simulink model "heatdrive_ecc_coupled_se21"  (R2025b)
settings: Solver=ode23t  StartTime=0.0  StopTime=10  FixedStep=0.1  MaxStep=0.4  RelTol=1e-2  AbsTol=1e-3
values from neighbouring files (symbols this model uses):
  cold_load_heat_W = 0.0    (= 0)    [Build_Simulink_Exchange_Params.m]
  cold_load_T_init = get_stage_field(stage_config, 'cold_load_T_in', get_stage_field(stage_config,          'chip_T_in', get_option_field(exchange_options, 'cold_load_T_init', get_option_field(exchange_options, 'chip_T_init', 293.0))))    [Build_Simulink_Exchange_Params.m]    (also in Create_Simulink_Exchange_Runtime.m = get_option_field(options, 'cold_load_T_init',          get_o)
  cold_sink_T_init = get_stage_field(stage_config, 'cold_sink_T_in', get_option_field(exchange_options, 'cold_sink_T_init', 293.0))    [Build_Simulink_Exchange_Params.m]    (also in Create_Simulink_Exchange_Runtime.m = get_option_field(options, 'cold_sink_T_init', ambient_T_init)
  hot_sink_T_init = get_stage_field(stage_config, 'hot_sink_T_in', get_option_field(exchange_options, 'hot_sink_T_init', 293.0))    [Build_Simulink_Exchange_Params.m]    (also in Create_Simulink_Exchange_Runtime.m = get_option_field(options, 'hot_sink_T_init', ambient_T_init))
  mdot_cooldown_source_kgps = mdot_target_kgps    [Build_Simulink_Exchange_Params.m]
  mdot_hold_source_kgps = mdot_target_kgps    [Build_Simulink_Exchange_Params.m]
  pressure_pi_bias_MPa = pressure_pi_dp_guess_MPa    [Build_Simulink_Exchange_Params.m]
  pressure_pi_error_filter_tau_s = max(get_option_field(exchange_options, 'pressure_pi_error_filter_tau_s', 0.002), 1.0e-5)    [Build_Simulink_Exchange_Params.m]
  pressure_pi_error_normalization_gain_kgps_inv = 1.0    (= 1)    [Build_Simulink_Exchange_Params.m]
  pressure_pi_max_MPa = pressure_pi_dp_guess_MPa + pressure_pi_margin_MPa    [Build_Simulink_Exchange_Params.m]
  shex_sink_T_init = get_option_field(exchange_options, 'shex_sink_T_init', hot_sink_T_init)    [Build_Simulink_Exchange_Params.m]
undefined symbols (not defined in the file or in its folder): constitutive_sample_time_s, constitutive_state21_initial, se_constitutive_T21_initial, se_pressure_integrator_max_MPa, se_pressure_pi_ki_MPa_per_kgps_s, se_pressure_pi_kp_MPa_per_kgps, se_pressure_pi_min_MPa, se_solver_T_init_21_internal, se_stage2_pressure_integrator_min_MPa, se_stage4_pressure_integrator_min_MPa, sma_constitutive_T21_initial, sma_mdot_stage1_source_kgps, sma_mdot_stage3_source_kgps, sma_pressure_integrator_max_MPa, sma_pressure_integrator_min_MPa, sma_pressure_pi_ki_MPa_per_kgps_s, sma_pressure_pi_kp_MPa_per_kgps, sma_pressure_pi_min_MPa, sma_solver_T_init_21_internal
libraries: fl_lib x484, nesl_utility x232, SimscapeFluids_lib x20
(part 4 of 8)

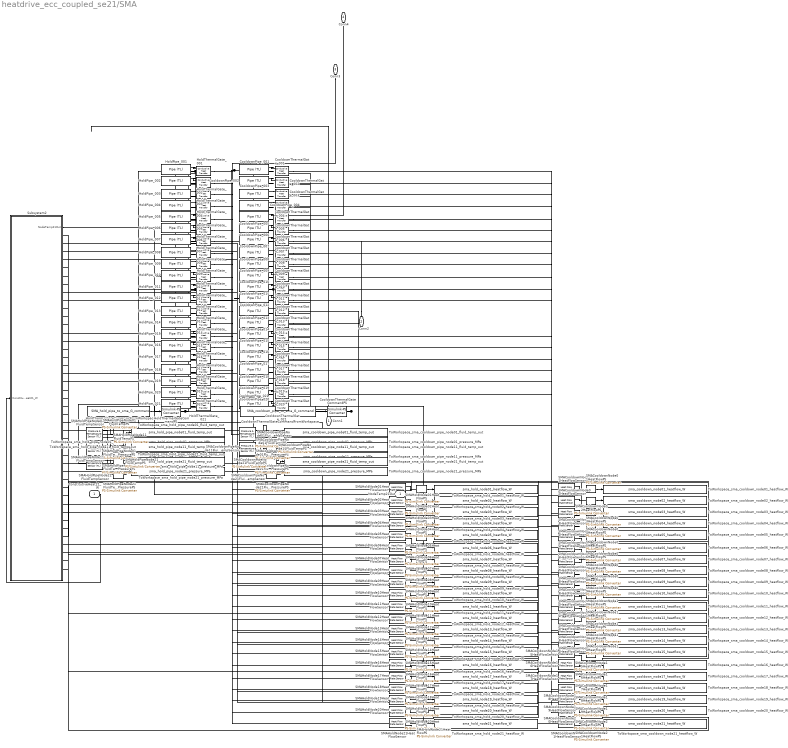
== system heatdrive_ecc_coupled_se21/SMA ==
  ConstitutiveHeat21_W : Inport
  CooldownPipe_001 : fl_lib/Thermal Liquid/Elements/Pipe (TL)  length=sma_article_pipe_segment_l m  area=sma_article_pipe_fa m^2  Dh=sma_article_pipe_Dh m  length_add=0 m  roughness=15e-6 m  Re_lam=2000  Re_tur=4000  shape_factor=64  Nu_lam=sma_article_Nu  dynamic_compressibility=false  inertia=false  p0=1 MPa  T0=sma_cooldown_fluid_T_init K  mdot0=0 kg/s  p_nominal=1 MPa  T_nominal=293.15 K
  CooldownPipe_002 : fl_lib/Thermal Liquid/Elements/Pipe (TL)  length=sma_article_pipe_segment_l m  area=sma_article_pipe_fa m^2  Dh=sma_article_pipe_Dh m  length_add=0 m  roughness=15e-6 m  Re_lam=2000  Re_tur=4000  shape_factor=64  Nu_lam=sma_article_Nu  dynamic_compressibility=false  inertia=false  p0=1 MPa  T0=sma_cooldown_fluid_T_init K  mdot0=0 kg/s  p_nominal=1 MPa  T_nominal=293.15 K
  CooldownPipe_003 : fl_lib/Thermal Liquid/Elements/Pipe (TL)  length=sma_article_pipe_segment_l m  area=sma_article_pipe_fa m^2  Dh=sma_article_pipe_Dh m  length_add=0 m  roughness=15e-6 m  Re_lam=2000  Re_tur=4000  shape_factor=64  Nu_lam=sma_article_Nu  dynamic_compressibility=false  inertia=false  p0=1 MPa  T0=sma_cooldown_fluid_T_init K  mdot0=0 kg/s  p_nominal=1 MPa  T_nominal=293.15 K
  CooldownPipe_004 : fl_lib/Thermal Liquid/Elements/Pipe (TL)  length=sma_article_pipe_segment_l m  area=sma_article_pipe_fa m^2  Dh=sma_article_pipe_Dh m  length_add=0 m  roughness=15e-6 m  Re_lam=2000  Re_tur=4000  shape_factor=64  Nu_lam=sma_article_Nu  dynamic_compressibility=false  inertia=false  p0=1 MPa  T0=sma_cooldown_fluid_T_init K  mdot0=0 kg/s  p_nominal=1 MPa  T_nominal=293.15 K
  CooldownPipe_005 : fl_lib/Thermal Liquid/Elements/Pipe (TL)  length=sma_article_pipe_segment_l m  area=sma_article_pipe_fa m^2  Dh=sma_article_pipe_Dh m  length_add=0 m  roughness=15e-6 m  Re_lam=2000  Re_tur=4000  shape_factor=64  Nu_lam=sma_article_Nu  dynamic_compressibility=false  inertia=false  p0=1 MPa  T0=sma_cooldown_fluid_T_init K  mdot0=0 kg/s  p_nominal=1 MPa  T_nominal=293.15 K
  CooldownPipe_006 : fl_lib/Thermal Liquid/Elements/Pipe (TL)  length=sma_article_pipe_segment_l m  area=sma_article_pipe_fa m^2  Dh=sma_article_pipe_Dh m  length_add=0 m  roughness=15e-6 m  Re_lam=2000  Re_tur=4000  shape_factor=64  Nu_lam=sma_article_Nu  dynamic_compressibility=false  inertia=false  p0=1 MPa  T0=sma_cooldown_fluid_T_init K  mdot0=0 kg/s  p_nominal=1 MPa  T_nominal=293.15 K
  CooldownPipe_007 : fl_lib/Thermal Liquid/Elements/Pipe (TL)  length=sma_article_pipe_segment_l m  area=sma_article_pipe_fa m^2  Dh=sma_article_pipe_Dh m  length_add=0 m  roughness=15e-6 m  Re_lam=2000  Re_tur=4000  shape_factor=64  Nu_lam=sma_article_Nu  dynamic_compressibility=false  inertia=false  p0=1 MPa  T0=sma_cooldown_fluid_T_init K  mdot0=0 kg/s  p_nominal=1 MPa  T_nominal=293.15 K
  CooldownPipe_008 : fl_lib/Thermal Liquid/Elements/Pipe (TL)  length=sma_article_pipe_segment_l m  area=sma_article_pipe_fa m^2  Dh=sma_article_pipe_Dh m  length_add=0 m  roughness=15e-6 m  Re_lam=2000  Re_tur=4000  shape_factor=64  Nu_lam=sma_article_Nu  dynamic_compressibility=false  inertia=false  p0=1 MPa  T0=sma_cooldown_fluid_T_init K  mdot0=0 kg/s  p_nominal=1 MPa  T_nominal=293.15 K
  CooldownPipe_009 : fl_lib/Thermal Liquid/Elements/Pipe (TL)  length=sma_article_pipe_segment_l m  area=sma_article_pipe_fa m^2  Dh=sma_article_pipe_Dh m  length_add=0 m  roughness=15e-6 m  Re_lam=2000  Re_tur=4000  shape_factor=64  Nu_lam=sma_article_Nu  dynamic_compressibility=false  inertia=false  p0=1 MPa  T0=sma_cooldown_fluid_T_init K  mdot0=0 kg/s  p_nominal=1 MPa  T_nominal=293.15 K
  CooldownPipe_010 : fl_lib/Thermal Liquid/Elements/Pipe (TL)  length=sma_article_pipe_segment_l m  area=sma_article_pipe_fa m^2  Dh=sma_article_pipe_Dh m  length_add=0 m  roughness=15e-6 m  Re_lam=2000  Re_tur=4000  shape_factor=64  Nu_lam=sma_article_Nu  dynamic_compressibility=false  inertia=false  p0=1 MPa  T0=sma_cooldown_fluid_T_init K  mdot0=0 kg/s  p_nominal=1 MPa  T_nominal=293.15 K
  CooldownPipe_011 : fl_lib/Thermal Liquid/Elements/Pipe (TL)  length=sma_article_pipe_segment_l m  area=sma_article_pipe_fa m^2  Dh=sma_article_pipe_Dh m  length_add=0 m  roughness=15e-6 m  Re_lam=2000  Re_tur=4000  shape_factor=64  Nu_lam=sma_article_Nu  dynamic_compressibility=false  inertia=false  p0=1 MPa  T0=sma_cooldown_fluid_T_init K  mdot0=0 kg/s  p_nominal=1 MPa  T_nominal=293.15 K
  CooldownPipe_012 : fl_lib/Thermal Liquid/Elements/Pipe (TL)  length=sma_article_pipe_segment_l m  area=sma_article_pipe_fa m^2  Dh=sma_article_pipe_Dh m  length_add=0 m  roughness=15e-6 m  Re_lam=2000  Re_tur=4000  shape_factor=64  Nu_lam=sma_article_Nu  dynamic_compressibility=false  inertia=false  p0=1 MPa  T0=sma_cooldown_fluid_T_init K  mdot0=0 kg/s  p_nominal=1 MPa  T_nominal=293.15 K
  CooldownPipe_013 : fl_lib/Thermal Liquid/Elements/Pipe (TL)  length=sma_article_pipe_segment_l m  area=sma_article_pipe_fa m^2  Dh=sma_article_pipe_Dh m  length_add=0 m  roughness=15e-6 m  Re_lam=2000  Re_tur=4000  shape_factor=64  Nu_lam=sma_article_Nu  dynamic_compressibility=false  inertia=false  p0=1 MPa  T0=sma_cooldown_fluid_T_init K  mdot0=0 kg/s  p_nominal=1 MPa  T_nominal=293.15 K
  CooldownPipe_014 : fl_lib/Thermal Liquid/Elements/Pipe (TL)  length=sma_article_pipe_segment_l m  area=sma_article_pipe_fa m^2  Dh=sma_article_pipe_Dh m  length_add=0 m  roughness=15e-6 m  Re_lam=2000  Re_tur=4000  shape_factor=64  Nu_lam=sma_article_Nu  dynamic_compressibility=false  inertia=false  p0=1 MPa  T0=sma_cooldown_fluid_T_init K  mdot0=0 kg/s  p_nominal=1 MPa  T_nominal=293.15 K
  CooldownPipe_015 : fl_lib/Thermal Liquid/Elements/Pipe (TL)  length=sma_article_pipe_segment_l m  area=sma_article_pipe_fa m^2  Dh=sma_article_pipe_Dh m  length_add=0 m  roughness=15e-6 m  Re_lam=2000  Re_tur=4000  shape_factor=64  Nu_lam=sma_article_Nu  dynamic_compressibility=false  inertia=false  p0=1 MPa  T0=sma_cooldown_fluid_T_init K  mdot0=0 kg/s  p_nominal=1 MPa  T_nominal=293.15 K
  CooldownPipe_016 : fl_lib/Thermal Liquid/Elements/Pipe (TL)  length=sma_article_pipe_segment_l m  area=sma_article_pipe_fa m^2  Dh=sma_article_pipe_Dh m  length_add=0 m  roughness=15e-6 m  Re_lam=2000  Re_tur=4000  shape_factor=64  Nu_lam=sma_article_Nu  dynamic_compressibility=false  inertia=false  p0=1 MPa  T0=sma_cooldown_fluid_T_init K  mdot0=0 kg/s  p_nominal=1 MPa  T_nominal=293.15 K
  CooldownPipe_017 : fl_lib/Thermal Liquid/Elements/Pipe (TL)  length=sma_article_pipe_segment_l m  area=sma_article_pipe_fa m^2  Dh=sma_article_pipe_Dh m  length_add=0 m  roughness=15e-6 m  Re_lam=2000  Re_tur=4000  shape_factor=64  Nu_lam=sma_article_Nu  dynamic_compressibility=false  inertia=false  p0=1 MPa  T0=sma_cooldown_fluid_T_init K  mdot0=0 kg/s  p_nominal=1 MPa  T_nominal=293.15 K
  CooldownPipe_018 : fl_lib/Thermal Liquid/Elements/Pipe (TL)  length=sma_article_pipe_segment_l m  area=sma_article_pipe_fa m^2  Dh=sma_article_pipe_Dh m  length_add=0 m  roughness=15e-6 m  Re_lam=2000  Re_tur=4000  shape_factor=64  Nu_lam=sma_article_Nu  dynamic_compressibility=false  inertia=false  p0=1 MPa  T0=sma_cooldown_fluid_T_init K  mdot0=0 kg/s  p_nominal=1 MPa  T_nominal=293.15 K
  CooldownPipe_019 : fl_lib/Thermal Liquid/Elements/Pipe (TL)  length=sma_article_pipe_segment_l m  area=sma_article_pipe_fa m^2  Dh=sma_article_pipe_Dh m  length_add=0 m  roughness=15e-6 m  Re_lam=2000  Re_tur=4000  shape_factor=64  Nu_lam=sma_article_Nu  dynamic_compressibility=false  inertia=false  p0=1 MPa  T0=sma_cooldown_fluid_T_init K  mdot0=0 kg/s  p_nominal=1 MPa  T_nominal=293.15 K
  CooldownPipe_020 : fl_lib/Thermal Liquid/Elements/Pipe (TL)  length=sma_article_pipe_segment_l m  area=sma_article_pipe_fa m^2  Dh=sma_article_pipe_Dh m  length_add=0 m  roughness=15e-6 m  Re_lam=2000  Re_tur=4000  shape_factor=64  Nu_lam=sma_article_Nu  dynamic_compressibility=false  inertia=false  p0=1 MPa  T0=sma_cooldown_fluid_T_init K  mdot0=0 kg/s  p_nominal=1 MPa  T_nominal=293.15 K
  CooldownPipe_021 : fl_lib/Thermal Liquid/Elements/Pipe (TL)  length=sma_article_pipe_segment_l m  area=sma_article_pipe_fa m^2  Dh=sma_article_pipe_Dh m  length_add=0 m  roughness=15e-6 m  Re_lam=2000  Re_tur=4000  shape_factor=64  Nu_lam=sma_article_Nu  dynamic_compressibility=false  inertia=false  p0=1 MPa  T0=sma_cooldown_fluid_T_init K  mdot0=0 kg/s  p_nominal=1 MPa  T_nominal=293.15 K
  CooldownThermalGateCommandFromWorkspace : FromWorkspace  VariableName=SMA_cooldown_pipe_to_sma_G_command  Interpolate=off  OutputAfterFinalValue=Holding final value
  CooldownThermalGateCommandPS : nesl_utility/Simulink-PS Converter  PhysicalDomain=network_engine_domain  SubClassName=ps_input  LeftPortType=input  RightPortType=output  PseudoPeriodic=off  Frequencies=[]  NoiseDistribution=none  NoiseParameters=[]  Unit=W/(K*m)  AffineConversion=off  FilteringAndDerivatives=provide  SimscapeFilterOrder=1  InputFilterTimeConstant=0.001  UdotUserProvided=0
  CooldownThermalGate_001 : fl_lib/Thermal/Thermal Elements/Conductive Heat Transfer  thermal_type=foundation.enum.ConstantVariableTabulated.Variable  wall_geometry=foundation.enum.ConductionWallGeometry.Planar  area=sma_pipe_fa m^2  thickness=1 m  d_in=0.05 m  d_out=0.1 m  L=1 m  th_cond_min=thermal_gate_min_conductivity_W_per_mK W/(K*m)  th_cond=sma_cooldown_pipe_to_sma_G_W_per_K W/(K*m)  th_cond_TLU=[413, 401, 392, 383, 371, 357, 342] W/(K*m)  temp_TLU=[200, 273, 400, 600, 800, 1000, 1200] K  T_specify=off  T_priority=None  T=0 K  T_nominal_specify=off  T_nominal_value=1  T_nominal_unit=K  Q_specify=off  Q_priority=None  Q=0 W  Q_nominal_specify=off  Q_nominal_value=1  Q_nominal_unit=W
      settings: InternalSimscapePortConfiguration="{\"Bottom\":[],\"Left\":[{\"id\":\"A\",\"label\":\"A\",\"type\":\"foundation.thermal.thermal\"},{\"id\":\"var_th_cond\",\"label\":\"K\",\"type\":\"input\"}],\"Right\":[{\"id\":\"B\",\"label\":\"B\",\"type\":\"foundation.thermal.thermal\"}],\"Top\":[]}"
  CooldownThermalGate_002 : fl_lib/Thermal/Thermal Elements/Conductive Heat Transfer  thermal_type=foundation.enum.ConstantVariableTabulated.Variable  wall_geometry=foundation.enum.ConductionWallGeometry.Planar  area=sma_pipe_fa m^2  thickness=1 m  d_in=0.05 m  d_out=0.1 m  L=1 m  th_cond_min=thermal_gate_min_conductivity_W_per_mK W/(K*m)  th_cond=sma_cooldown_pipe_to_sma_G_W_per_K W/(K*m)  th_cond_TLU=[413, 401, 392, 383, 371, 357, 342] W/(K*m)  temp_TLU=[200, 273, 400, 600, 800, 1000, 1200] K  T_specify=off  T_priority=None  T=0 K  T_nominal_specify=off  T_nominal_value=1  T_nominal_unit=K  Q_specify=off  Q_priority=None  Q=0 W  Q_nominal_specify=off  Q_nominal_value=1  Q_nominal_unit=W
      settings: InternalSimscapePortConfiguration="{\"Bottom\":[],\"Left\":[{\"id\":\"A\",\"label\":\"A\",\"type\":\"foundation.thermal.thermal\"},{\"id\":\"var_th_cond\",\"label\":\"K\",\"type\":\"input\"}],\"Right\":[{\"id\":\"B\",\"label\":\"B\",\"type\":\"foundation.thermal.thermal\"}],\"Top\":[]}"
  CooldownThermalGate_003 : fl_lib/Thermal/Thermal Elements/Conductive Heat Transfer  thermal_type=foundation.enum.ConstantVariableTabulated.Variable  wall_geometry=foundation.enum.ConductionWallGeometry.Planar  area=sma_pipe_fa m^2  thickness=1 m  d_in=0.05 m  d_out=0.1 m  L=1 m  th_cond_min=thermal_gate_min_conductivity_W_per_mK W/(K*m)  th_cond=sma_cooldown_pipe_to_sma_G_W_per_K W/(K*m)  th_cond_TLU=[413, 401, 392, 383, 371, 357, 342] W/(K*m)  temp_TLU=[200, 273, 400, 600, 800, 1000, 1200] K  T_specify=off  T_priority=None  T=0 K  T_nominal_specify=off  T_nominal_value=1  T_nominal_unit=K  Q_specify=off  Q_priority=None  Q=0 W  Q_nominal_specify=off  Q_nominal_value=1  Q_nominal_unit=W
      settings: InternalSimscapePortConfiguration="{\"Bottom\":[],\"Left\":[{\"id\":\"A\",\"label\":\"A\",\"type\":\"foundation.thermal.thermal\"},{\"id\":\"var_th_cond\",\"label\":\"K\",\"type\":\"input\"}],\"Right\":[{\"id\":\"B\",\"label\":\"B\",\"type\":\"foundation.thermal.thermal\"}],\"Top\":[]}"
  CooldownThermalGate_004 : fl_lib/Thermal/Thermal Elements/Conductive Heat Transfer  thermal_type=foundation.enum.ConstantVariableTabulated.Variable  wall_geometry=foundation.enum.ConductionWallGeometry.Planar  area=sma_pipe_fa m^2  thickness=1 m  d_in=0.05 m  d_out=0.1 m  L=1 m  th_cond_min=thermal_gate_min_conductivity_W_per_mK W/(K*m)  th_cond=sma_cooldown_pipe_to_sma_G_W_per_K W/(K*m)  th_cond_TLU=[413, 401, 392, 383, 371, 357, 342] W/(K*m)  temp_TLU=[200, 273, 400, 600, 800, 1000, 1200] K  T_specify=off  T_priority=None  T=0 K  T_nominal_specify=off  T_nominal_value=1  T_nominal_unit=K  Q_specify=off  Q_priority=None  Q=0 W  Q_nominal_specify=off  Q_nominal_value=1  Q_nominal_unit=W
      settings: InternalSimscapePortConfiguration="{\"Bottom\":[],\"Left\":[{\"id\":\"A\",\"label\":\"A\",\"type\":\"foundation.thermal.thermal\"},{\"id\":\"var_th_cond\",\"label\":\"K\",\"type\":\"input\"}],\"Right\":[{\"id\":\"B\",\"label\":\"B\",\"type\":\"foundation.thermal.thermal\"}],\"Top\":[]}"
  CooldownThermalGate_005 : fl_lib/Thermal/Thermal Elements/Conductive Heat Transfer  thermal_type=foundation.enum.ConstantVariableTabulated.Variable  wall_geometry=foundation.enum.ConductionWallGeometry.Planar  area=sma_pipe_fa m^2  thickness=1 m  d_in=0.05 m  d_out=0.1 m  L=1 m  th_cond_min=thermal_gate_min_conductivity_W_per_mK W/(K*m)  th_cond=sma_cooldown_pipe_to_sma_G_W_per_K W/(K*m)  th_cond_TLU=[413, 401, 392, 383, 371, 357, 342] W/(K*m)  temp_TLU=[200, 273, 400, 600, 800, 1000, 1200] K  T_specify=off  T_priority=None  T=0 K  T_nominal_specify=off  T_nominal_value=1  T_nominal_unit=K  Q_specify=off  Q_priority=None  Q=0 W  Q_nominal_specify=off  Q_nominal_value=1  Q_nominal_unit=W
      settings: InternalSimscapePortConfiguration="{\"Bottom\":[],\"Left\":[{\"id\":\"A\",\"label\":\"A\",\"type\":\"foundation.thermal.thermal\"},{\"id\":\"var_th_cond\",\"label\":\"K\",\"type\":\"input\"}],\"Right\":[{\"id\":\"B\",\"label\":\"B\",\"type\":\"foundation.thermal.thermal\"}],\"Top\":[]}"
  CooldownThermalGate_006 : fl_lib/Thermal/Thermal Elements/Conductive Heat Transfer  thermal_type=foundation.enum.ConstantVariableTabulated.Variable  wall_geometry=foundation.enum.ConductionWallGeometry.Planar  area=sma_pipe_fa m^2  thickness=1 m  d_in=0.05 m  d_out=0.1 m  L=1 m  th_cond_min=thermal_gate_min_conductivity_W_per_mK W/(K*m)  th_cond=sma_cooldown_pipe_to_sma_G_W_per_K W/(K*m)  th_cond_TLU=[413, 401, 392, 383, 371, 357, 342] W/(K*m)  temp_TLU=[200, 273, 400, 600, 800, 1000, 1200] K  T_specify=off  T_priority=None  T=0 K  T_nominal_specify=off  T_nominal_value=1  T_nominal_unit=K  Q_specify=off  Q_priority=None  Q=0 W  Q_nominal_specify=off  Q_nominal_value=1  Q_nominal_unit=W
      settings: InternalSimscapePortConfiguration="{\"Bottom\":[],\"Left\":[{\"id\":\"A\",\"label\":\"A\",\"type\":\"foundation.thermal.thermal\"},{\"id\":\"var_th_cond\",\"label\":\"K\",\"type\":\"input\"}],\"Right\":[{\"id\":\"B\",\"label\":\"B\",\"type\":\"foundation.thermal.thermal\"}],\"Top\":[]}"
  CooldownThermalGate_007 : fl_lib/Thermal/Thermal Elements/Conductive Heat Transfer  thermal_type=foundation.enum.ConstantVariableTabulated.Variable  wall_geometry=foundation.enum.ConductionWallGeometry.Planar  area=sma_pipe_fa m^2  thickness=1 m  d_in=0.05 m  d_out=0.1 m  L=1 m  th_cond_min=thermal_gate_min_conductivity_W_per_mK W/(K*m)  th_cond=sma_cooldown_pipe_to_sma_G_W_per_K W/(K*m)  th_cond_TLU=[413, 401, 392, 383, 371, 357, 342] W/(K*m)  temp_TLU=[200, 273, 400, 600, 800, 1000, 1200] K  T_specify=off  T_priority=None  T=0 K  T_nominal_specify=off  T_nominal_value=1  T_nominal_unit=K  Q_specify=off  Q_priority=None  Q=0 W  Q_nominal_specify=off  Q_nominal_value=1  Q_nominal_unit=W
      settings: InternalSimscapePortConfiguration="{\"Bottom\":[],\"Left\":[{\"id\":\"A\",\"label\":\"A\",\"type\":\"foundation.thermal.thermal\"},{\"id\":\"var_th_cond\",\"label\":\"K\",\"type\":\"input\"}],\"Right\":[{\"id\":\"B\",\"label\":\"B\",\"type\":\"foundation.thermal.thermal\"}],\"Top\":[]}"
  CooldownThermalGate_008 : fl_lib/Thermal/Thermal Elements/Conductive Heat Transfer  thermal_type=foundation.enum.ConstantVariableTabulated.Variable  wall_geometry=foundation.enum.ConductionWallGeometry.Planar  area=sma_pipe_fa m^2  thickness=1 m  d_in=0.05 m  d_out=0.1 m  L=1 m  th_cond_min=thermal_gate_min_conductivity_W_per_mK W/(K*m)  th_cond=sma_cooldown_pipe_to_sma_G_W_per_K W/(K*m)  th_cond_TLU=[413, 401, 392, 383, 371, 357, 342] W/(K*m)  temp_TLU=[200, 273, 400, 600, 800, 1000, 1200] K  T_specify=off  T_priority=None  T=0 K  T_nominal_specify=off  T_nominal_value=1  T_nominal_unit=K  Q_specify=off  Q_priority=None  Q=0 W  Q_nominal_specify=off  Q_nominal_value=1  Q_nominal_unit=W
      settings: InternalSimscapePortConfiguration="{\"Bottom\":[],\"Left\":[{\"id\":\"A\",\"label\":\"A\",\"type\":\"foundation.thermal.thermal\"},{\"id\":\"var_th_cond\",\"label\":\"K\",\"type\":\"input\"}],\"Right\":[{\"id\":\"B\",\"label\":\"B\",\"type\":\"foundation.thermal.thermal\"}],\"Top\":[]}"
  CooldownThermalGate_009 : fl_lib/Thermal/Thermal Elements/Conductive Heat Transfer  thermal_type=foundation.enum.ConstantVariableTabulated.Variable  wall_geometry=foundation.enum.ConductionWallGeometry.Planar  area=sma_pipe_fa m^2  thickness=1 m  d_in=0.05 m  d_out=0.1 m  L=1 m  th_cond_min=thermal_gate_min_conductivity_W_per_mK W/(K*m)  th_cond=sma_cooldown_pipe_to_sma_G_W_per_K W/(K*m)  th_cond_TLU=[413, 401, 392, 383, 371, 357, 342] W/(K*m)  temp_TLU=[200, 273, 400, 600, 800, 1000, 1200] K  T_specify=off  T_priority=None  T=0 K  T_nominal_specify=off  T_nominal_value=1  T_nominal_unit=K  Q_specify=off  Q_priority=None  Q=0 W  Q_nominal_specify=off  Q_nominal_value=1  Q_nominal_unit=W
      settings: InternalSimscapePortConfiguration="{\"Bottom\":[],\"Left\":[{\"id\":\"A\",\"label\":\"A\",\"type\":\"foundation.thermal.thermal\"},{\"id\":\"var_th_cond\",\"label\":\"K\",\"type\":\"input\"}],\"Right\":[{\"id\":\"B\",\"label\":\"B\",\"type\":\"foundation.thermal.thermal\"}],\"Top\":[]}"
  CooldownThermalGate_010 : fl_lib/Thermal/Thermal Elements/Conductive Heat Transfer  thermal_type=foundation.enum.ConstantVariableTabulated.Variable  wall_geometry=foundation.enum.ConductionWallGeometry.Planar  area=sma_pipe_fa m^2  thickness=1 m  d_in=0.05 m  d_out=0.1 m  L=1 m  th_cond_min=thermal_gate_min_conductivity_W_per_mK W/(K*m)  th_cond=sma_cooldown_pipe_to_sma_G_W_per_K W/(K*m)  th_cond_TLU=[413, 401, 392, 383, 371, 357, 342] W/(K*m)  temp_TLU=[200, 273, 400, 600, 800, 1000, 1200] K  T_specify=off  T_priority=None  T=0 K  T_nominal_specify=off  T_nominal_value=1  T_nominal_unit=K  Q_specify=off  Q_priority=None  Q=0 W  Q_nominal_specify=off  Q_nominal_value=1  Q_nominal_unit=W
      settings: InternalSimscapePortConfiguration="{\"Bottom\":[],\"Left\":[{\"id\":\"A\",\"label\":\"A\",\"type\":\"foundation.thermal.thermal\"},{\"id\":\"var_th_cond\",\"label\":\"K\",\"type\":\"input\"}],\"Right\":[{\"id\":\"B\",\"label\":\"B\",\"type\":\"foundation.thermal.thermal\"}],\"Top\":[]}"
  CooldownThermalGate_011 : fl_lib/Thermal/Thermal Elements/Conductive Heat Transfer  thermal_type=foundation.enum.ConstantVariableTabulated.Variable  wall_geometry=foundation.enum.ConductionWallGeometry.Planar  area=sma_pipe_fa m^2  thickness=1 m  d_in=0.05 m  d_out=0.1 m  L=1 m  th_cond_min=thermal_gate_min_conductivity_W_per_mK W/(K*m)  th_cond=sma_cooldown_pipe_to_sma_G_W_per_K W/(K*m)  th_cond_TLU=[413, 401, 392, 383, 371, 357, 342] W/(K*m)  temp_TLU=[200, 273, 400, 600, 800, 1000, 1200] K  T_specify=off  T_priority=None  T=0 K  T_nominal_specify=off  T_nominal_value=1  T_nominal_unit=K  Q_specify=off  Q_priority=None  Q=0 W  Q_nominal_specify=off  Q_nominal_value=1  Q_nominal_unit=W
      settings: InternalSimscapePortConfiguration="{\"Bottom\":[],\"Left\":[{\"id\":\"A\",\"label\":\"A\",\"type\":\"foundation.thermal.thermal\"},{\"id\":\"var_th_cond\",\"label\":\"K\",\"type\":\"input\"}],\"Right\":[{\"id\":\"B\",\"label\":\"B\",\"type\":\"foundation.thermal.thermal\"}],\"Top\":[]}"
  CooldownThermalGate_012 : fl_lib/Thermal/Thermal Elements/Conductive Heat Transfer  thermal_type=foundation.enum.ConstantVariableTabulated.Variable  wall_geometry=foundation.enum.ConductionWallGeometry.Planar  area=sma_pipe_fa m^2  thickness=1 m  d_in=0.05 m  d_out=0.1 m  L=1 m  th_cond_min=thermal_gate_min_conductivity_W_per_mK W/(K*m)  th_cond=sma_cooldown_pipe_to_sma_G_W_per_K W/(K*m)  th_cond_TLU=[413, 401, 392, 383, 371, 357, 342] W/(K*m)  temp_TLU=[200, 273, 400, 600, 800, 1000, 1200] K  T_specify=off  T_priority=None  T=0 K  T_nominal_specify=off  T_nominal_value=1  T_nominal_unit=K  Q_specify=off  Q_priority=None  Q=0 W  Q_nominal_specify=off  Q_nominal_value=1  Q_nominal_unit=W
      settings: InternalSimscapePortConfiguration="{\"Bottom\":[],\"Left\":[{\"id\":\"A\",\"label\":\"A\",\"type\":\"foundation.thermal.thermal\"},{\"id\":\"var_th_cond\",\"label\":\"K\",\"type\":\"input\"}],\"Right\":[{\"id\":\"B\",\"label\":\"B\",\"type\":\"foundation.thermal.thermal\"}],\"Top\":[]}"
  CooldownThermalGate_013 : fl_lib/Thermal/Thermal Elements/Conductive Heat Transfer  thermal_type=foundation.enum.ConstantVariableTabulated.Variable  wall_geometry=foundation.enum.ConductionWallGeometry.Planar  area=sma_pipe_fa m^2  thickness=1 m  d_in=0.05 m  d_out=0.1 m  L=1 m  th_cond_min=thermal_gate_min_conductivity_W_per_mK W/(K*m)  th_cond=sma_cooldown_pipe_to_sma_G_W_per_K W/(K*m)  th_cond_TLU=[413, 401, 392, 383, 371, 357, 342] W/(K*m)  temp_TLU=[200, 273, 400, 600, 800, 1000, 1200] K  T_specify=off  T_priority=None  T=0 K  T_nominal_specify=off  T_nominal_value=1  T_nominal_unit=K  Q_specify=off  Q_priority=None  Q=0 W  Q_nominal_specify=off  Q_nominal_value=1  Q_nominal_unit=W
      settings: InternalSimscapePortConfiguration="{\"Bottom\":[],\"Left\":[{\"id\":\"A\",\"label\":\"A\",\"type\":\"foundation.thermal.thermal\"},{\"id\":\"var_th_cond\",\"label\":\"K\",\"type\":\"input\"}],\"Right\":[{\"id\":\"B\",\"label\":\"B\",\"type\":\"foundation.thermal.thermal\"}],\"Top\":[]}"
  CooldownThermalGate_014 : fl_lib/Thermal/Thermal Elements/Conductive Heat Transfer  thermal_type=foundation.enum.ConstantVariableTabulated.Variable  wall_geometry=foundation.enum.ConductionWallGeometry.Planar  area=sma_pipe_fa m^2  thickness=1 m  d_in=0.05 m  d_out=0.1 m  L=1 m  th_cond_min=thermal_gate_min_conductivity_W_per_mK W/(K*m)  th_cond=sma_cooldown_pipe_to_sma_G_W_per_K W/(K*m)  th_cond_TLU=[413, 401, 392, 383, 371, 357, 342] W/(K*m)  temp_TLU=[200, 273, 400, 600, 800, 1000, 1200] K  T_specify=off  T_priority=None  T=0 K  T_nominal_specify=off  T_nominal_value=1  T_nominal_unit=K  Q_specify=off  Q_priority=None  Q=0 W  Q_nominal_specify=off  Q_nominal_value=1  Q_nominal_unit=W
      settings: InternalSimscapePortConfiguration="{\"Bottom\":[],\"Left\":[{\"id\":\"A\",\"label\":\"A\",\"type\":\"foundation.thermal.thermal\"},{\"id\":\"var_th_cond\",\"label\":\"K\",\"type\":\"input\"}],\"Right\":[{\"id\":\"B\",\"label\":\"B\",\"type\":\"foundation.thermal.thermal\"}],\"Top\":[]}"
  CooldownThermalGate_015 : fl_lib/Thermal/Thermal Elements/Conductive Heat Transfer  thermal_type=foundation.enum.ConstantVariableTabulated.Variable  wall_geometry=foundation.enum.ConductionWallGeometry.Planar  area=sma_pipe_fa m^2  thickness=1 m  d_in=0.05 m  d_out=0.1 m  L=1 m  th_cond_min=thermal_gate_min_conductivity_W_per_mK W/(K*m)  th_cond=sma_cooldown_pipe_to_sma_G_W_per_K W/(K*m)  th_cond_TLU=[413, 401, 392, 383, 371, 357, 342] W/(K*m)  temp_TLU=[200, 273, 400, 600, 800, 1000, 1200] K  T_specify=off  T_priority=None  T=0 K  T_nominal_specify=off  T_nominal_value=1  T_nominal_unit=K  Q_specify=off  Q_priority=None  Q=0 W  Q_nominal_specify=off  Q_nominal_value=1  Q_nominal_unit=W
      settings: InternalSimscapePortConfiguration="{\"Bottom\":[],\"Left\":[{\"id\":\"A\",\"label\":\"A\",\"type\":\"foundation.thermal.thermal\"},{\"id\":\"var_th_cond\",\"label\":\"K\",\"type\":\"input\"}],\"Right\":[{\"id\":\"B\",\"label\":\"B\",\"type\":\"foundation.thermal.thermal\"}],\"Top\":[]}"
  CooldownThermalGate_016 : fl_lib/Thermal/Thermal Elements/Conductive Heat Transfer  thermal_type=foundation.enum.ConstantVariableTabulated.Variable  wall_geometry=foundation.enum.ConductionWallGeometry.Planar  area=sma_pipe_fa m^2  thickness=1 m  d_in=0.05 m  d_out=0.1 m  L=1 m  th_cond_min=thermal_gate_min_conductivity_W_per_mK W/(K*m)  th_cond=sma_cooldown_pipe_to_sma_G_W_per_K W/(K*m)  th_cond_TLU=[413, 401, 392, 383, 371, 357, 342] W/(K*m)  temp_TLU=[200, 273, 400, 600, 800, 1000, 1200] K  T_specify=off  T_priority=None  T=0 K  T_nominal_specify=off  T_nominal_value=1  T_nominal_unit=K  Q_specify=off  Q_priority=None  Q=0 W  Q_nominal_specify=off  Q_nominal_value=1  Q_nominal_unit=W
      settings: InternalSimscapePortConfiguration="{\"Bottom\":[],\"Left\":[{\"id\":\"A\",\"label\":\"A\",\"type\":\"foundation.thermal.thermal\"},{\"id\":\"var_th_cond\",\"label\":\"K\",\"type\":\"input\"}],\"Right\":[{\"id\":\"B\",\"label\":\"B\",\"type\":\"foundation.thermal.thermal\"}],\"Top\":[]}"
  CooldownThermalGate_017 : fl_lib/Thermal/Thermal Elements/Conductive Heat Transfer  thermal_type=foundation.enum.ConstantVariableTabulated.Variable  wall_geometry=foundation.enum.ConductionWallGeometry.Planar  area=sma_pipe_fa m^2  thickness=1 m  d_in=0.05 m  d_out=0.1 m  L=1 m  th_cond_min=thermal_gate_min_conductivity_W_per_mK W/(K*m)  th_cond=sma_cooldown_pipe_to_sma_G_W_per_K W/(K*m)  th_cond_TLU=[413, 401, 392, 383, 371, 357, 342] W/(K*m)  temp_TLU=[200, 273, 400, 600, 800, 1000, 1200] K  T_specify=off  T_priority=None  T=0 K  T_nominal_specify=off  T_nominal_value=1  T_nominal_unit=K  Q_specify=off  Q_priority=None  Q=0 W  Q_nominal_specify=off  Q_nominal_value=1  Q_nominal_unit=W
      settings: InternalSimscapePortConfiguration="{\"Bottom\":[],\"Left\":[{\"id\":\"A\",\"label\":\"A\",\"type\":\"foundation.thermal.thermal\"},{\"id\":\"var_th_cond\",\"label\":\"K\",\"type\":\"input\"}],\"Right\":[{\"id\":\"B\",\"label\":\"B\",\"type\":\"foundation.thermal.thermal\"}],\"Top\":[]}"
  CooldownThermalGate_018 : fl_lib/Thermal/Thermal Elements/Conductive Heat Transfer  thermal_type=foundation.enum.ConstantVariableTabulated.Variable  wall_geometry=foundation.enum.ConductionWallGeometry.Planar  area=sma_pipe_fa m^2  thickness=1 m  d_in=0.05 m  d_out=0.1 m  L=1 m  th_cond_min=thermal_gate_min_conductivity_W_per_mK W/(K*m)  th_cond=sma_cooldown_pipe_to_sma_G_W_per_K W/(K*m)  th_cond_TLU=[413, 401, 392, 383, 371, 357, 342] W/(K*m)  temp_TLU=[200, 273, 400, 600, 800, 1000, 1200] K  T_specify=off  T_priority=None  T=0 K  T_nominal_specify=off  T_nominal_value=1  T_nominal_unit=K  Q_specify=off  Q_priority=None  Q=0 W  Q_nominal_specify=off  Q_nominal_value=1  Q_nominal_unit=W
      settings: InternalSimscapePortConfiguration="{\"Bottom\":[],\"Left\":[{\"id\":\"A\",\"label\":\"A\",\"type\":\"foundation.thermal.thermal\"},{\"id\":\"var_th_cond\",\"label\":\"K\",\"type\":\"input\"}],\"Right\":[{\"id\":\"B\",\"label\":\"B\",\"type\":\"foundation.thermal.thermal\"}],\"Top\":[]}"
  CooldownThermalGate_019 : fl_lib/Thermal/Thermal Elements/Conductive Heat Transfer  thermal_type=foundation.enum.ConstantVariableTabulated.Variable  wall_geometry=foundation.enum.ConductionWallGeometry.Planar  area=sma_pipe_fa m^2  thickness=1 m  d_in=0.05 m  d_out=0.1 m  L=1 m  th_cond_min=thermal_gate_min_conductivity_W_per_mK W/(K*m)  th_cond=sma_cooldown_pipe_to_sma_G_W_per_K W/(K*m)  th_cond_TLU=[413, 401, 392, 383, 371, 357, 342] W/(K*m)  temp_TLU=[200, 273, 400, 600, 800, 1000, 1200] K  T_specify=off  T_priority=None  T=0 K  T_nominal_specify=off  T_nominal_value=1  T_nominal_unit=K  Q_specify=off  Q_priority=None  Q=0 W  Q_nominal_specify=off  Q_nominal_value=1  Q_nominal_unit=W
      settings: InternalSimscapePortConfiguration="{\"Bottom\":[],\"Left\":[{\"id\":\"A\",\"label\":\"A\",\"type\":\"foundation.thermal.thermal\"},{\"id\":\"var_th_cond\",\"label\":\"K\",\"type\":\"input\"}],\"Right\":[{\"id\":\"B\",\"label\":\"B\",\"type\":\"foundation.thermal.thermal\"}],\"Top\":[]}"
  CooldownThermalGate_020 : fl_lib/Thermal/Thermal Elements/Conductive Heat Transfer  thermal_type=foundation.enum.ConstantVariableTabulated.Variable  wall_geometry=foundation.enum.ConductionWallGeometry.Planar  area=sma_pipe_fa m^2  thickness=1 m  d_in=0.05 m  d_out=0.1 m  L=1 m  th_cond_min=thermal_gate_min_conductivity_W_per_mK W/(K*m)  th_cond=sma_cooldown_pipe_to_sma_G_W_per_K W/(K*m)  th_cond_TLU=[413, 401, 392, 383, 371, 357, 342] W/(K*m)  temp_TLU=[200, 273, 400, 600, 800, 1000, 1200] K  T_specify=off  T_priority=None  T=0 K  T_nominal_specify=off  T_nominal_value=1  T_nominal_unit=K  Q_specify=off  Q_priority=None  Q=0 W  Q_nominal_specify=off  Q_nominal_value=1  Q_nominal_unit=W
      settings: InternalSimscapePortConfiguration="{\"Bottom\":[],\"Left\":[{\"id\":\"A\",\"label\":\"A\",\"type\":\"foundation.thermal.thermal\"},{\"id\":\"var_th_cond\",\"label\":\"K\",\"type\":\"input\"}],\"Right\":[{\"id\":\"B\",\"label\":\"B\",\"type\":\"foundation.thermal.thermal\"}],\"Top\":[]}"
  CooldownThermalGate_021 : fl_lib/Thermal/Thermal Elements/Conductive Heat Transfer  thermal_type=foundation.enum.ConstantVariableTabulated.Variable  wall_geometry=foundation.enum.ConductionWallGeometry.Planar  area=sma_pipe_fa m^2  thickness=1 m  d_in=0.05 m  d_out=0.1 m  L=1 m  th_cond_min=thermal_gate_min_conductivity_W_per_mK W/(K*m)  th_cond=sma_cooldown_pipe_to_sma_G_W_per_K W/(K*m)  th_cond_TLU=[413, 401, 392, 383, 371, 357, 342] W/(K*m)  temp_TLU=[200, 273, 400, 600, 800, 1000, 1200] K  T_specify=off  T_priority=None  T=0 K  T_nominal_specify=off  T_nominal_value=1  T_nominal_unit=K  Q_specify=off  Q_priority=None  Q=0 W  Q_nominal_specify=off  Q_nominal_value=1  Q_nominal_unit=W
      settings: InternalSimscapePortConfiguration="{\"Bottom\":[],\"Left\":[{\"id\":\"A\",\"label\":\"A\",\"type\":\"foundation.thermal.thermal\"},{\"id\":\"var_th_cond\",\"label\":\"K\",\"type\":\"input\"}],\"Right\":[{\"id\":\"B\",\"label\":\"B\",\"type\":\"foundation.thermal.thermal\"}],\"Top\":[]}"
  HoldPipe_001 : fl_lib/Thermal Liquid/Elements/Pipe (TL)  length=sma_article_pipe_segment_l m  area=sma_article_pipe_fa m^2  Dh=sma_article_pipe_Dh m  length_add=0 m  roughness=15e-6 m  Re_lam=2000  Re_tur=4000  shape_factor=64  Nu_lam=sma_article_Nu  dynamic_compressibility=false  inertia=false  p0=1 MPa  T0=sma_hold_fluid_T_init K  mdot0=0 kg/s  p_nominal=1 MPa  T_nominal=293.15 K
  HoldPipe_002 : fl_lib/Thermal Liquid/Elements/Pipe (TL)  length=sma_article_pipe_segment_l m  area=sma_article_pipe_fa m^2  Dh=sma_article_pipe_Dh m  length_add=0 m  roughness=15e-6 m  Re_lam=2000  Re_tur=4000  shape_factor=64  Nu_lam=sma_article_Nu  dynamic_compressibility=false  inertia=false  p0=1 MPa  T0=sma_hold_fluid_T_init K  mdot0=0 kg/s  p_nominal=1 MPa  T_nominal=293.15 K
  HoldPipe_003 : fl_lib/Thermal Liquid/Elements/Pipe (TL)  length=sma_article_pipe_segment_l m  area=sma_article_pipe_fa m^2  Dh=sma_article_pipe_Dh m  length_add=0 m  roughness=15e-6 m  Re_lam=2000  Re_tur=4000  shape_factor=64  Nu_lam=sma_article_Nu  dynamic_compressibility=false  inertia=false  p0=1 MPa  T0=sma_hold_fluid_T_init K  mdot0=0 kg/s  p_nominal=1 MPa  T_nominal=293.15 K
  HoldPipe_004 : fl_lib/Thermal Liquid/Elements/Pipe (TL)  length=sma_article_pipe_segment_l m  area=sma_article_pipe_fa m^2  Dh=sma_article_pipe_Dh m  length_add=0 m  roughness=15e-6 m  Re_lam=2000  Re_tur=4000  shape_factor=64  Nu_lam=sma_article_Nu  dynamic_compressibility=false  inertia=false  p0=1 MPa  T0=sma_hold_fluid_T_init K  mdot0=0 kg/s  p_nominal=1 MPa  T_nominal=293.15 K
  HoldPipe_005 : fl_lib/Thermal Liquid/Elements/Pipe (TL)  length=sma_article_pipe_segment_l m  area=sma_article_pipe_fa m^2  Dh=sma_article_pipe_Dh m  length_add=0 m  roughness=15e-6 m  Re_lam=2000  Re_tur=4000  shape_factor=64  Nu_lam=sma_article_Nu  dynamic_compressibility=false  inertia=false  p0=1 MPa  T0=sma_hold_fluid_T_init K  mdot0=0 kg/s  p_nominal=1 MPa  T_nominal=293.15 K
  HoldPipe_006 : fl_lib/Thermal Liquid/Elements/Pipe (TL)  length=sma_article_pipe_segment_l m  area=sma_article_pipe_fa m^2  Dh=sma_article_pipe_Dh m  length_add=0 m  roughness=15e-6 m  Re_lam=2000  Re_tur=4000  shape_factor=64  Nu_lam=sma_article_Nu  dynamic_compressibility=false  inertia=false  p0=1 MPa  T0=sma_hold_fluid_T_init K  mdot0=0 kg/s  p_nominal=1 MPa  T_nominal=293.15 K
  HoldPipe_007 : fl_lib/Thermal Liquid/Elements/Pipe (TL)  length=sma_article_pipe_segment_l m  area=sma_article_pipe_fa m^2  Dh=sma_article_pipe_Dh m  length_add=0 m  roughness=15e-6 m  Re_lam=2000  Re_tur=4000  shape_factor=64  Nu_lam=sma_article_Nu  dynamic_compressibility=false  inertia=false  p0=1 MPa  T0=sma_hold_fluid_T_init K  mdot0=0 kg/s  p_nominal=1 MPa  T_nominal=293.15 K
  HoldPipe_008 : fl_lib/Thermal Liquid/Elements/Pipe (TL)  length=sma_article_pipe_segment_l m  area=sma_article_pipe_fa m^2  Dh=sma_article_pipe_Dh m  length_add=0 m  roughness=15e-6 m  Re_lam=2000  Re_tur=4000  shape_factor=64  Nu_lam=sma_article_Nu  dynamic_compressibility=false  inertia=false  p0=1 MPa  T0=sma_hold_fluid_T_init K  mdot0=0 kg/s  p_nominal=1 MPa  T_nominal=293.15 K
  HoldPipe_009 : fl_lib/Thermal Liquid/Elements/Pipe (TL)  length=sma_article_pipe_segment_l m  area=sma_article_pipe_fa m^2  Dh=sma_article_pipe_Dh m  length_add=0 m  roughness=15e-6 m  Re_lam=2000  Re_tur=4000  shape_factor=64  Nu_lam=sma_article_Nu  dynamic_compressibility=false  inertia=false  p0=1 MPa  T0=sma_hold_fluid_T_init K  mdot0=0 kg/s  p_nominal=1 MPa  T_nominal=293.15 K
  HoldPipe_010 : fl_lib/Thermal Liquid/Elements/Pipe (TL)  length=sma_article_pipe_segment_l m  area=sma_article_pipe_fa m^2  Dh=sma_article_pipe_Dh m  length_add=0 m  roughness=15e-6 m  Re_lam=2000  Re_tur=4000  shape_factor=64  Nu_lam=sma_article_Nu  dynamic_compressibility=false  inertia=false  p0=1 MPa  T0=sma_hold_fluid_T_init K  mdot0=0 kg/s  p_nominal=1 MPa  T_nominal=293.15 K
  HoldPipe_011 : fl_lib/Thermal Liquid/Elements/Pipe (TL)  length=sma_article_pipe_segment_l m  area=sma_article_pipe_fa m^2  Dh=sma_article_pipe_Dh m  length_add=0 m  roughness=15e-6 m  Re_lam=2000  Re_tur=4000  shape_factor=64  Nu_lam=sma_article_Nu  dynamic_compressibility=false  inertia=false  p0=1 MPa  T0=sma_hold_fluid_T_init K  mdot0=0 kg/s  p_nominal=1 MPa  T_nominal=293.15 K
  HoldPipe_012 : fl_lib/Thermal Liquid/Elements/Pipe (TL)  length=sma_article_pipe_segment_l m  area=sma_article_pipe_fa m^2  Dh=sma_article_pipe_Dh m  length_add=0 m  roughness=15e-6 m  Re_lam=2000  Re_tur=4000  shape_factor=64  Nu_lam=sma_article_Nu  dynamic_compressibility=false  inertia=false  p0=1 MPa  T0=sma_hold_fluid_T_init K  mdot0=0 kg/s  p_nominal=1 MPa  T_nominal=293.15 K
  HoldPipe_013 : fl_lib/Thermal Liquid/Elements/Pipe (TL)  length=sma_article_pipe_segment_l m  area=sma_article_pipe_fa m^2  Dh=sma_article_pipe_Dh m  length_add=0 m  roughness=15e-6 m  Re_lam=2000  Re_tur=4000  shape_factor=64  Nu_lam=sma_article_Nu  dynamic_compressibility=false  inertia=false  p0=1 MPa  T0=sma_hold_fluid_T_init K  mdot0=0 kg/s  p_nominal=1 MPa  T_nominal=293.15 K
  HoldPipe_014 : fl_lib/Thermal Liquid/Elements/Pipe (TL)  length=sma_article_pipe_segment_l m  area=sma_article_pipe_fa m^2  Dh=sma_article_pipe_Dh m  length_add=0 m  roughness=15e-6 m  Re_lam=2000  Re_tur=4000  shape_factor=64  Nu_lam=sma_article_Nu  dynamic_compressibility=false  inertia=false  p0=1 MPa  T0=sma_hold_fluid_T_init K  mdot0=0 kg/s  p_nominal=1 MPa  T_nominal=293.15 K
  HoldPipe_015 : fl_lib/Thermal Liquid/Elements/Pipe (TL)  length=sma_article_pipe_segment_l m  area=sma_article_pipe_fa m^2  Dh=sma_article_pipe_Dh m  length_add=0 m  roughness=15e-6 m  Re_lam=2000  Re_tur=4000  shape_factor=64  Nu_lam=sma_article_Nu  dynamic_compressibility=false  inertia=false  p0=1 MPa  T0=sma_hold_fluid_T_init K  mdot0=0 kg/s  p_nominal=1 MPa  T_nominal=293.15 K
  HoldPipe_016 : fl_lib/Thermal Liquid/Elements/Pipe (TL)  length=sma_article_pipe_segment_l m  area=sma_article_pipe_fa m^2  Dh=sma_article_pipe_Dh m  length_add=0 m  roughness=15e-6 m  Re_lam=2000  Re_tur=4000  shape_factor=64  Nu_lam=sma_article_Nu  dynamic_compressibility=false  inertia=false  p0=1 MPa  T0=sma_hold_fluid_T_init K  mdot0=0 kg/s  p_nominal=1 MPa  T_nominal=293.15 K
  HoldPipe_017 : fl_lib/Thermal Liquid/Elements/Pipe (TL)  length=sma_article_pipe_segment_l m  area=sma_article_pipe_fa m^2  Dh=sma_article_pipe_Dh m  length_add=0 m  roughness=15e-6 m  Re_lam=2000  Re_tur=4000  shape_factor=64  Nu_lam=sma_article_Nu  dynamic_compressibility=false  inertia=false  p0=1 MPa  T0=sma_hold_fluid_T_init K  mdot0=0 kg/s  p_nominal=1 MPa  T_nominal=293.15 K
  HoldPipe_018 : fl_lib/Thermal Liquid/Elements/Pipe (TL)  length=sma_article_pipe_segment_l m  area=sma_article_pipe_fa m^2  Dh=sma_article_pipe_Dh m  length_add=0 m  roughness=15e-6 m  Re_lam=2000  Re_tur=4000  shape_factor=64  Nu_lam=sma_article_Nu  dynamic_compressibility=false  inertia=false  p0=1 MPa  T0=sma_hold_fluid_T_init K  mdot0=0 kg/s  p_nominal=1 MPa  T_nominal=293.15 K
  HoldPipe_019 : fl_lib/Thermal Liquid/Elements/Pipe (TL)  length=sma_article_pipe_segment_l m  area=sma_article_pipe_fa m^2  Dh=sma_article_pipe_Dh m  length_add=0 m  roughness=15e-6 m  Re_lam=2000  Re_tur=4000  shape_factor=64  Nu_lam=sma_article_Nu  dynamic_compressibility=false  inertia=false  p0=1 MPa  T0=sma_hold_fluid_T_init K  mdot0=0 kg/s  p_nominal=1 MPa  T_nominal=293.15 K
  HoldPipe_020 : fl_lib/Thermal Liquid/Elements/Pipe (TL)  length=sma_article_pipe_segment_l m  area=sma_article_pipe_fa m^2  Dh=sma_article_pipe_Dh m  length_add=0 m  roughness=15e-6 m  Re_lam=2000  Re_tur=4000  shape_factor=64  Nu_lam=sma_article_Nu  dynamic_compressibility=false  inertia=false  p0=1 MPa  T0=sma_hold_fluid_T_init K  mdot0=0 kg/s  p_nominal=1 MPa  T_nominal=293.15 K
  HoldPipe_021 : fl_lib/Thermal Liquid/Elements/Pipe (TL)  length=sma_article_pipe_segment_l m  area=sma_article_pipe_fa m^2  Dh=sma_article_pipe_Dh m  length_add=0 m  roughness=15e-6 m  Re_lam=2000  Re_tur=4000  shape_factor=64  Nu_lam=sma_article_Nu  dynamic_compressibility=false  inertia=false  p0=1 MPa  T0=sma_hold_fluid_T_init K  mdot0=0 kg/s  p_nominal=1 MPa  T_nominal=293.15 K
  HoldThermalGateCommandFromWorkspace : FromWorkspace  VariableName=SMA_hold_pipe_to_sma_G_command  Interpolate=off  OutputAfterFinalValue=Holding final value
  HoldThermalGateCommandPS : nesl_utility/Simulink-PS Converter  PhysicalDomain=network_engine_domain  SubClassName=ps_input  LeftPortType=input  RightPortType=output  PseudoPeriodic=off  Frequencies=[]  NoiseDistribution=none  NoiseParameters=[]  Unit=W/(K*m)  AffineConversion=off  FilteringAndDerivatives=provide  SimscapeFilterOrder=1  InputFilterTimeConstant=0.001  UdotUserProvided=0
  HoldThermalGate_001 : fl_lib/Thermal/Thermal Elements/Conductive Heat Transfer  thermal_type=foundation.enum.ConstantVariableTabulated.Variable  wall_geometry=foundation.enum.ConductionWallGeometry.Planar  area=sma_pipe_fa m^2  thickness=1 m  d_in=0.05 m  d_out=0.1 m  L=1 m  th_cond_min=thermal_gate_min_conductivity_W_per_mK W/(K*m)  th_cond=sma_hold_pipe_to_sma_G_W_per_K W/(K*m)  th_cond_TLU=[413, 401, 392, 383, 371, 357, 342] W/(K*m)  temp_TLU=[200, 273, 400, 600, 800, 1000, 1200] K  T_specify=off  T_priority=None  T=0 K  T_nominal_specify=off  T_nominal_value=1  T_nominal_unit=K  Q_specify=off  Q_priority=None  Q=0 W  Q_nominal_specify=off  Q_nominal_value=1  Q_nominal_unit=W
      settings: InternalSimscapePortConfiguration="{\"Bottom\":[],\"Left\":[{\"id\":\"A\",\"label\":\"A\",\"type\":\"foundation.thermal.thermal\"},{\"id\":\"var_th_cond\",\"label\":\"K\",\"type\":\"input\"}],\"Right\":[{\"id\":\"B\",\"label\":\"B\",\"type\":\"foundation.thermal.thermal\"}],\"Top\":[]}"
  HoldThermalGate_002 : fl_lib/Thermal/Thermal Elements/Conductive Heat Transfer  thermal_type=foundation.enum.ConstantVariableTabulated.Variable  wall_geometry=foundation.enum.ConductionWallGeometry.Planar  area=sma_pipe_fa m^2  thickness=1 m  d_in=0.05 m  d_out=0.1 m  L=1 m  th_cond_min=thermal_gate_min_conductivity_W_per_mK W/(K*m)  th_cond=sma_hold_pipe_to_sma_G_W_per_K W/(K*m)  th_cond_TLU=[413, 401, 392, 383, 371, 357, 342] W/(K*m)  temp_TLU=[200, 273, 400, 600, 800, 1000, 1200] K  T_specify=off  T_priority=None  T=0 K  T_nominal_specify=off  T_nominal_value=1  T_nominal_unit=K  Q_specify=off  Q_priority=None  Q=0 W  Q_nominal_specify=off  Q_nominal_value=1  Q_nominal_unit=W
      settings: InternalSimscapePortConfiguration="{\"Bottom\":[],\"Left\":[{\"id\":\"A\",\"label\":\"A\",\"type\":\"foundation.thermal.thermal\"},{\"id\":\"var_th_cond\",\"label\":\"K\",\"type\":\"input\"}],\"Right\":[{\"id\":\"B\",\"label\":\"B\",\"type\":\"foundation.thermal.thermal\"}],\"Top\":[]}"
  HoldThermalGate_003 : fl_lib/Thermal/Thermal Elements/Conductive Heat Transfer  thermal_type=foundation.enum.ConstantVariableTabulated.Variable  wall_geometry=foundation.enum.ConductionWallGeometry.Planar  area=sma_pipe_fa m^2  thickness=1 m  d_in=0.05 m  d_out=0.1 m  L=1 m  th_cond_min=thermal_gate_min_conductivity_W_per_mK W/(K*m)  th_cond=sma_hold_pipe_to_sma_G_W_per_K W/(K*m)  th_cond_TLU=[413, 401, 392, 383, 371, 357, 342] W/(K*m)  temp_TLU=[200, 273, 400, 600, 800, 1000, 1200] K  T_specify=off  T_priority=None  T=0 K  T_nominal_specify=off  T_nominal_value=1  T_nominal_unit=K  Q_specify=off  Q_priority=None  Q=0 W  Q_nominal_specify=off  Q_nominal_value=1  Q_nominal_unit=W
      settings: InternalSimscapePortConfiguration="{\"Bottom\":[],\"Left\":[{\"id\":\"A\",\"label\":\"A\",\"type\":\"foundation.thermal.thermal\"},{\"id\":\"var_th_cond\",\"label\":\"K\",\"type\":\"input\"}],\"Right\":[{\"id\":\"B\",\"label\":\"B\",\"type\":\"foundation.thermal.thermal\"}],\"Top\":[]}"
  HoldThermalGate_004 : fl_lib/Thermal/Thermal Elements/Conductive Heat Transfer  thermal_type=foundation.enum.ConstantVariableTabulated.Variable  wall_geometry=foundation.enum.ConductionWallGeometry.Planar  area=sma_pipe_fa m^2  thickness=1 m  d_in=0.05 m  d_out=0.1 m  L=1 m  th_cond_min=thermal_gate_min_conductivity_W_per_mK W/(K*m)  th_cond=sma_hold_pipe_to_sma_G_W_per_K W/(K*m)  th_cond_TLU=[413, 401, 392, 383, 371, 357, 342] W/(K*m)  temp_TLU=[200, 273, 400, 600, 800, 1000, 1200] K  T_specify=off  T_priority=None  T=0 K  T_nominal_specify=off  T_nominal_value=1  T_nominal_unit=K  Q_specify=off  Q_priority=None  Q=0 W  Q_nominal_specify=off  Q_nominal_value=1  Q_nominal_unit=W
      settings: InternalSimscapePortConfiguration="{\"Bottom\":[],\"Left\":[{\"id\":\"A\",\"label\":\"A\",\"type\":\"foundation.thermal.thermal\"},{\"id\":\"var_th_cond\",\"label\":\"K\",\"type\":\"input\"}],\"Right\":[{\"id\":\"B\",\"label\":\"B\",\"type\":\"foundation.thermal.thermal\"}],\"Top\":[]}"
  HoldThermalGate_005 : fl_lib/Thermal/Thermal Elements/Conductive Heat Transfer  thermal_type=foundation.enum.ConstantVariableTabulated.Variable  wall_geometry=foundation.enum.ConductionWallGeometry.Planar  area=sma_pipe_fa m^2  thickness=1 m  d_in=0.05 m  d_out=0.1 m  L=1 m  th_cond_min=thermal_gate_min_conductivity_W_per_mK W/(K*m)  th_cond=sma_hold_pipe_to_sma_G_W_per_K W/(K*m)  th_cond_TLU=[413, 401, 392, 383, 371, 357, 342] W/(K*m)  temp_TLU=[200, 273, 400, 600, 800, 1000, 1200] K  T_specify=off  T_priority=None  T=0 K  T_nominal_specify=off  T_nominal_value=1  T_nominal_unit=K  Q_specify=off  Q_priority=None  Q=0 W  Q_nominal_specify=off  Q_nominal_value=1  Q_nominal_unit=W
      settings: InternalSimscapePortConfiguration="{\"Bottom\":[],\"Left\":[{\"id\":\"A\",\"label\":\"A\",\"type\":\"foundation.thermal.thermal\"},{\"id\":\"var_th_cond\",\"label\":\"K\",\"type\":\"input\"}],\"Right\":[{\"id\":\"B\",\"label\":\"B\",\"type\":\"foundation.thermal.thermal\"}],\"Top\":[]}"
  HoldThermalGate_006 : fl_lib/Thermal/Thermal Elements/Conductive Heat Transfer  thermal_type=foundation.enum.ConstantVariableTabulated.Variable  wall_geometry=foundation.enum.ConductionWallGeometry.Planar  area=sma_pipe_fa m^2  thickness=1 m  d_in=0.05 m  d_out=0.1 m  L=1 m  th_cond_min=thermal_gate_min_conductivity_W_per_mK W/(K*m)  th_cond=sma_hold_pipe_to_sma_G_W_per_K W/(K*m)  th_cond_TLU=[413, 401, 392, 383, 371, 357, 342] W/(K*m)  temp_TLU=[200, 273, 400, 600, 800, 1000, 1200] K  T_specify=off  T_priority=None  T=0 K  T_nominal_specify=off  T_nominal_value=1  T_nominal_unit=K  Q_specify=off  Q_priority=None  Q=0 W  Q_nominal_specify=off  Q_nominal_value=1  Q_nominal_unit=W
      settings: InternalSimscapePortConfiguration="{\"Bottom\":[],\"Left\":[{\"id\":\"A\",\"label\":\"A\",\"type\":\"foundation.thermal.thermal\"},{\"id\":\"var_th_cond\",\"label\":\"K\",\"type\":\"input\"}],\"Right\":[{\"id\":\"B\",\"label\":\"B\",\"type\":\"foundation.thermal.thermal\"}],\"Top\":[]}"
  HoldThermalGate_007 : fl_lib/Thermal/Thermal Elements/Conductive Heat Transfer  thermal_type=foundation.enum.ConstantVariableTabulated.Variable  wall_geometry=foundation.enum.ConductionWallGeometry.Planar  area=sma_pipe_fa m^2  thickness=1 m  d_in=0.05 m  d_out=0.1 m  L=1 m  th_cond_min=thermal_gate_min_conductivity_W_per_mK W/(K*m)  th_cond=sma_hold_pipe_to_sma_G_W_per_K W/(K*m)  th_cond_TLU=[413, 401, 392, 383, 371, 357, 342] W/(K*m)  temp_TLU=[200, 273, 400, 600, 800, 1000, 1200] K  T_specify=off  T_priority=None  T=0 K  T_nominal_specify=off  T_nominal_value=1  T_nominal_unit=K  Q_specify=off  Q_priority=None  Q=0 W  Q_nominal_specify=off  Q_nominal_value=1  Q_nominal_unit=W
      settings: InternalSimscapePortConfiguration="{\"Bottom\":[],\"Left\":[{\"id\":\"A\",\"label\":\"A\",\"type\":\"foundation.thermal.thermal\"},{\"id\":\"var_th_cond\",\"label\":\"K\",\"type\":\"input\"}],\"Right\":[{\"id\":\"B\",\"label\":\"B\",\"type\":\"foundation.thermal.thermal\"}],\"Top\":[]}"
  HoldThermalGate_008 : fl_lib/Thermal/Thermal Elements/Conductive Heat Transfer  thermal_type=foundation.enum.ConstantVariableTabulated.Variable  wall_geometry=foundation.enum.ConductionWallGeometry.Planar  area=sma_pipe_fa m^2  thickness=1 m  d_in=0.05 m  d_out=0.1 m  L=1 m  th_cond_min=thermal_gate_min_conductivity_W_per_mK W/(K*m)  th_cond=sma_hold_pipe_to_sma_G_W_per_K W/(K*m)  th_cond_TLU=[413, 401, 392, 383, 371, 357, 342] W/(K*m)  temp_TLU=[200, 273, 400, 600, 800, 1000, 1200] K  T_specify=off  T_priority=None  T=0 K  T_nominal_specify=off  T_nominal_value=1  T_nominal_unit=K  Q_specify=off  Q_priority=None  Q=0 W  Q_nominal_specify=off  Q_nominal_value=1  Q_nominal_unit=W
      settings: InternalSimscapePortConfiguration="{\"Bottom\":[],\"Left\":[{\"id\":\"A\",\"label\":\"A\",\"type\":\"foundation.thermal.thermal\"},{\"id\":\"var_th_cond\",\"label\":\"K\",\"type\":\"input\"}],\"Right\":[{\"id\":\"B\",\"label\":\"B\",\"type\":\"foundation.thermal.thermal\"}],\"Top\":[]}"
  HoldThermalGate_009 : fl_lib/Thermal/Thermal Elements/Conductive Heat Transfer  thermal_type=foundation.enum.ConstantVariableTabulated.Variable  wall_geometry=foundation.enum.ConductionWallGeometry.Planar  area=sma_pipe_fa m^2  thickness=1 m  d_in=0.05 m  d_out=0.1 m  L=1 m  th_cond_min=thermal_gate_min_conductivity_W_per_mK W/(K*m)  th_cond=sma_hold_pipe_to_sma_G_W_per_K W/(K*m)  th_cond_TLU=[413, 401, 392, 383, 371, 357, 342] W/(K*m)  temp_TLU=[200, 273, 400, 600, 800, 1000, 1200] K  T_specify=off  T_priority=None  T=0 K  T_nominal_specify=off  T_nominal_value=1  T_nominal_unit=K  Q_specify=off  Q_priority=None  Q=0 W  Q_nominal_specify=off  Q_nominal_value=1  Q_nominal_unit=W
      settings: InternalSimscapePortConfiguration="{\"Bottom\":[],\"Left\":[{\"id\":\"A\",\"label\":\"A\",\"type\":\"foundation.thermal.thermal\"},{\"id\":\"var_th_cond\",\"label\":\"K\",\"type\":\"input\"}],\"Right\":[{\"id\":\"B\",\"label\":\"B\",\"type\":\"foundation.thermal.thermal\"}],\"Top\":[]}"
  HoldThermalGate_010 : fl_lib/Thermal/Thermal Elements/Conductive Heat Transfer  thermal_type=foundation.enum.ConstantVariableTabulated.Variable  wall_geometry=foundation.enum.ConductionWallGeometry.Planar  area=sma_pipe_fa m^2  thickness=1 m  d_in=0.05 m  d_out=0.1 m  L=1 m  th_cond_min=thermal_gate_min_conductivity_W_per_mK W/(K*m)  th_cond=sma_hold_pipe_to_sma_G_W_per_K W/(K*m)  th_cond_TLU=[413, 401, 392, 383, 371, 357, 342] W/(K*m)  temp_TLU=[200, 273, 400, 600, 800, 1000, 1200] K  T_specify=off  T_priority=None  T=0 K  T_nominal_specify=off  T_nominal_value=1  T_nominal_unit=K  Q_specify=off  Q_priority=None  Q=0 W  Q_nominal_specify=off  Q_nominal_value=1  Q_nominal_unit=W
      settings: InternalSimscapePortConfiguration="{\"Bottom\":[],\"Left\":[{\"id\":\"A\",\"label\":\"A\",\"type\":\"foundation.thermal.thermal\"},{\"id\":\"var_th_cond\",\"label\":\"K\",\"type\":\"input\"}],\"Right\":[{\"id\":\"B\",\"label\":\"B\",\"type\":\"foundation.thermal.thermal\"}],\"Top\":[]}"
  HoldThermalGate_011 : fl_lib/Thermal/Thermal Elements/Conductive Heat Transfer  thermal_type=foundation.enum.ConstantVariableTabulated.Variable  wall_geometry=foundation.enum.ConductionWallGeometry.Planar  area=sma_pipe_fa m^2  thickness=1 m  d_in=0.05 m  d_out=0.1 m  L=1 m  th_cond_min=thermal_gate_min_conductivity_W_per_mK W/(K*m)  th_cond=sma_hold_pipe_to_sma_G_W_per_K W/(K*m)  th_cond_TLU=[413, 401, 392, 383, 371, 357, 342] W/(K*m)  temp_TLU=[200, 273, 400, 600, 800, 1000, 1200] K  T_specify=off  T_priority=None  T=0 K  T_nominal_specify=off  T_nominal_value=1  T_nominal_unit=K  Q_specify=off  Q_priority=None  Q=0 W  Q_nominal_specify=off  Q_nominal_value=1  Q_nominal_unit=W
      settings: InternalSimscapePortConfiguration="{\"Bottom\":[],\"Left\":[{\"id\":\"A\",\"label\":\"A\",\"type\":\"foundation.thermal.thermal\"},{\"id\":\"var_th_cond\",\"label\":\"K\",\"type\":\"input\"}],\"Right\":[{\"id\":\"B\",\"label\":\"B\",\"type\":\"foundation.thermal.thermal\"}],\"Top\":[]}"
  HoldThermalGate_012 : fl_lib/Thermal/Thermal Elements/Conductive Heat Transfer  thermal_type=foundation.enum.ConstantVariableTabulated.Variable  wall_geometry=foundation.enum.ConductionWallGeometry.Planar  area=sma_pipe_fa m^2  thickness=1 m  d_in=0.05 m  d_out=0.1 m  L=1 m  th_cond_min=thermal_gate_min_conductivity_W_per_mK W/(K*m)  th_cond=sma_hold_pipe_to_sma_G_W_per_K W/(K*m)  th_cond_TLU=[413, 401, 392, 383, 371, 357, 342] W/(K*m)  temp_TLU=[200, 273, 400, 600, 800, 1000, 1200] K  T_specify=off  T_priority=None  T=0 K  T_nominal_specify=off  T_nominal_value=1  T_nominal_unit=K  Q_specify=off  Q_priority=None  Q=0 W  Q_nominal_specify=off  Q_nominal_value=1  Q_nominal_unit=W
      settings: InternalSimscapePortConfiguration="{\"Bottom\":[],\"Left\":[{\"id\":\"A\",\"label\":\"A\",\"type\":\"foundation.thermal.thermal\"},{\"id\":\"var_th_cond\",\"label\":\"K\",\"type\":\"input\"}],\"Right\":[{\"id\":\"B\",\"label\":\"B\",\"type\":\"foundation.thermal.thermal\"}],\"Top\":[]}"
  HoldThermalGate_013 : fl_lib/Thermal/Thermal Elements/Conductive Heat Transfer  thermal_type=foundation.enum.ConstantVariableTabulated.Variable  wall_geometry=foundation.enum.ConductionWallGeometry.Planar  area=sma_pipe_fa m^2  thickness=1 m  d_in=0.05 m  d_out=0.1 m  L=1 m  th_cond_min=thermal_gate_min_conductivity_W_per_mK W/(K*m)  th_cond=sma_hold_pipe_to_sma_G_W_per_K W/(K*m)  th_cond_TLU=[413, 401, 392, 383, 371, 357, 342] W/(K*m)  temp_TLU=[200, 273, 400, 600, 800, 1000, 1200] K  T_specify=off  T_priority=None  T=0 K  T_nominal_specify=off  T_nominal_value=1  T_nominal_unit=K  Q_specify=off  Q_priority=None  Q=0 W  Q_nominal_specify=off  Q_nominal_value=1  Q_nominal_unit=W
      settings: InternalSimscapePortConfiguration="{\"Bottom\":[],\"Left\":[{\"id\":\"A\",\"label\":\"A\",\"type\":\"foundation.thermal.thermal\"},{\"id\":\"var_th_cond\",\"label\":\"K\",\"type\":\"input\"}],\"Right\":[{\"id\":\"B\",\"label\":\"B\",\"type\":\"foundation.thermal.thermal\"}],\"Top\":[]}"
  HoldThermalGate_014 : fl_lib/Thermal/Thermal Elements/Conductive Heat Transfer  thermal_type=foundation.enum.ConstantVariableTabulated.Variable  wall_geometry=foundation.enum.ConductionWallGeometry.Planar  area=sma_pipe_fa m^2  thickness=1 m  d_in=0.05 m  d_out=0.1 m  L=1 m  th_cond_min=thermal_gate_min_conductivity_W_per_mK W/(K*m)  th_cond=sma_hold_pipe_to_sma_G_W_per_K W/(K*m)  th_cond_TLU=[413, 401, 392, 383, 371, 357, 342] W/(K*m)  temp_TLU=[200, 273, 400, 600, 800, 1000, 1200] K  T_specify=off  T_priority=None  T=0 K  T_nominal_specify=off  T_nominal_value=1  T_nominal_unit=K  Q_specify=off  Q_priority=None  Q=0 W  Q_nominal_specify=off  Q_nominal_value=1  Q_nominal_unit=W
      settings: InternalSimscapePortConfiguration="{\"Bottom\":[],\"Left\":[{\"id\":\"A\",\"label\":\"A\",\"type\":\"foundation.thermal.thermal\"},{\"id\":\"var_th_cond\",\"label\":\"K\",\"type\":\"input\"}],\"Right\":[{\"id\":\"B\",\"label\":\"B\",\"type\":\"foundation.thermal.thermal\"}],\"Top\":[]}"
  HoldThermalGate_015 : fl_lib/Thermal/Thermal Elements/Conductive Heat Transfer  thermal_type=foundation.enum.ConstantVariableTabulated.Variable  wall_geometry=foundation.enum.ConductionWallGeometry.Planar  area=sma_pipe_fa m^2  thickness=1 m  d_in=0.05 m  d_out=0.1 m  L=1 m  th_cond_min=thermal_gate_min_conductivity_W_per_mK W/(K*m)  th_cond=sma_hold_pipe_to_sma_G_W_per_K W/(K*m)  th_cond_TLU=[413, 401, 392, 383, 371, 357, 342] W/(K*m)  temp_TLU=[200, 273, 400, 600, 800, 1000, 1200] K  T_specify=off  T_priority=None  T=0 K  T_nominal_specify=off  T_nominal_value=1  T_nominal_unit=K  Q_specify=off  Q_priority=None  Q=0 W  Q_nominal_specify=off  Q_nominal_value=1  Q_nominal_unit=W
      settings: InternalSimscapePortConfiguration="{\"Bottom\":[],\"Left\":[{\"id\":\"A\",\"label\":\"A\",\"type\":\"foundation.thermal.thermal\"},{\"id\":\"var_th_cond\",\"label\":\"K\",\"type\":\"input\"}],\"Right\":[{\"id\":\"B\",\"label\":\"B\",\"type\":\"foundation.thermal.thermal\"}],\"Top\":[]}"
  HoldThermalGate_016 : fl_lib/Thermal/Thermal Elements/Conductive Heat Transfer  thermal_type=foundation.enum.ConstantVariableTabulated.Variable  wall_geometry=foundation.enum.ConductionWallGeometry.Planar  area=sma_pipe_fa m^2  thickness=1 m  d_in=0.05 m  d_out=0.1 m  L=1 m  th_cond_min=thermal_gate_min_conductivity_W_per_mK W/(K*m)  th_cond=sma_hold_pipe_to_sma_G_W_per_K W/(K*m)  th_cond_TLU=[413, 401, 392, 383, 371, 357, 342] W/(K*m)  temp_TLU=[200, 273, 400, 600, 800, 1000, 1200] K  T_specify=off  T_priority=None  T=0 K  T_nominal_specify=off  T_nominal_value=1  T_nominal_unit=K  Q_specify=off  Q_priority=None  Q=0 W  Q_nominal_specify=off  Q_nominal_value=1  Q_nominal_unit=W
      settings: InternalSimscapePortConfiguration="{\"Bottom\":[],\"Left\":[{\"id\":\"A\",\"label\":\"A\",\"type\":\"foundation.thermal.thermal\"},{\"id\":\"var_th_cond\",\"label\":\"K\",\"type\":\"input\"}],\"Right\":[{\"id\":\"B\",\"label\":\"B\",\"type\":\"foundation.thermal.thermal\"}],\"Top\":[]}"
  HoldThermalGate_017 : fl_lib/Thermal/Thermal Elements/Conductive Heat Transfer  thermal_type=foundation.enum.ConstantVariableTabulated.Variable  wall_geometry=foundation.enum.ConductionWallGeometry.Planar  area=sma_pipe_fa m^2  thickness=1 m  d_in=0.05 m  d_out=0.1 m  L=1 m  th_cond_min=thermal_gate_min_conductivity_W_per_mK W/(K*m)  th_cond=sma_hold_pipe_to_sma_G_W_per_K W/(K*m)  th_cond_TLU=[413, 401, 392, 383, 371, 357, 342] W/(K*m)  temp_TLU=[200, 273, 400, 600, 800, 1000, 1200] K  T_specify=off  T_priority=None  T=0 K  T_nominal_specify=off  T_nominal_value=1  T_nominal_unit=K  Q_specify=off  Q_priority=None  Q=0 W  Q_nominal_specify=off  Q_nominal_value=1  Q_nominal_unit=W
      settings: InternalSimscapePortConfiguration="{\"Bottom\":[],\"Left\":[{\"id\":\"A\",\"label\":\"A\",\"type\":\"foundation.thermal.thermal\"},{\"id\":\"var_th_cond\",\"label\":\"K\",\"type\":\"input\"}],\"Right\":[{\"id\":\"B\",\"label\":\"B\",\"type\":\"foundation.thermal.thermal\"}],\"Top\":[]}"
  HoldThermalGate_018 : fl_lib/Thermal/Thermal Elements/Conductive Heat Transfer  thermal_type=foundation.enum.ConstantVariableTabulated.Variable  wall_geometry=foundation.enum.ConductionWallGeometry.Planar  area=sma_pipe_fa m^2  thickness=1 m  d_in=0.05 m  d_out=0.1 m  L=1 m  th_cond_min=thermal_gate_min_conductivity_W_per_mK W/(K*m)  th_cond=sma_hold_pipe_to_sma_G_W_per_K W/(K*m)  th_cond_TLU=[413, 401, 392, 383, 371, 357, 342] W/(K*m)  temp_TLU=[200, 273, 400, 600, 800, 1000, 1200] K  T_specify=off  T_priority=None  T=0 K  T_nominal_specify=off  T_nominal_value=1  T_nominal_unit=K  Q_specify=off  Q_priority=None  Q=0 W  Q_nominal_specify=off  Q_nominal_value=1  Q_nominal_unit=W
      settings: InternalSimscapePortConfiguration="{\"Bottom\":[],\"Left\":[{\"id\":\"A\",\"label\":\"A\",\"type\":\"foundation.thermal.thermal\"},{\"id\":\"var_th_cond\",\"label\":\"K\",\"type\":\"input\"}],\"Right\":[{\"id\":\"B\",\"label\":\"B\",\"type\":\"foundation.thermal.thermal\"}],\"Top\":[]}"
  HoldThermalGate_019 : fl_lib/Thermal/Thermal Elements/Conductive Heat Transfer  thermal_type=foundation.enum.ConstantVariableTabulated.Variable  wall_geometry=foundation.enum.ConductionWallGeometry.Planar  area=sma_pipe_fa m^2  thickness=1 m  d_in=0.05 m  d_out=0.1 m  L=1 m  th_cond_min=thermal_gate_min_conductivity_W_per_mK W/(K*m)  th_cond=sma_hold_pipe_to_sma_G_W_per_K W/(K*m)  th_cond_TLU=[413, 401, 392, 383, 371, 357, 342] W/(K*m)  temp_TLU=[200, 273, 400, 600, 800, 1000, 1200] K  T_specify=off  T_priority=None  T=0 K  T_nominal_specify=off  T_nominal_value=1  T_nominal_unit=K  Q_specify=off  Q_priority=None  Q=0 W  Q_nominal_specify=off  Q_nominal_value=1  Q_nominal_unit=W
      settings: InternalSimscapePortConfiguration="{\"Bottom\":[],\"Left\":[{\"id\":\"A\",\"label\":\"A\",\"type\":\"foundation.thermal.thermal\"},{\"id\":\"var_th_cond\",\"label\":\"K\",\"type\":\"input\"}],\"Right\":[{\"id\":\"B\",\"label\":\"B\",\"type\":\"foundation.thermal.thermal\"}],\"Top\":[]}"
  HoldThermalGate_020 : fl_lib/Thermal/Thermal Elements/Conductive Heat Transfer  thermal_type=foundation.enum.ConstantVariableTabulated.Variable  wall_geometry=foundation.enum.ConductionWallGeometry.Planar  area=sma_pipe_fa m^2  thickness=1 m  d_in=0.05 m  d_out=0.1 m  L=1 m  th_cond_min=thermal_gate_min_conductivity_W_per_mK W/(K*m)  th_cond=sma_hold_pipe_to_sma_G_W_per_K W/(K*m)  th_cond_TLU=[413, 401, 392, 383, 371, 357, 342] W/(K*m)  temp_TLU=[200, 273, 400, 600, 800, 1000, 1200] K  T_specify=off  T_priority=None  T=0 K  T_nominal_specify=off  T_nominal_value=1  T_nominal_unit=K  Q_specify=off  Q_priority=None  Q=0 W  Q_nominal_specify=off  Q_nominal_value=1  Q_nominal_unit=W
      settings: InternalSimscapePortConfiguration="{\"Bottom\":[],\"Left\":[{\"id\":\"A\",\"label\":\"A\",\"type\":\"foundation.thermal.thermal\"},{\"id\":\"var_th_cond\",\"label\":\"K\",\"type\":\"input\"}],\"Right\":[{\"id\":\"B\",\"label\":\"B\",\"type\":\"foundation.thermal.thermal\"}],\"Top\":[]}"
  HoldThermalGate_021 : fl_lib/Thermal/Thermal Elements/Conductive Heat Transfer  thermal_type=foundation.enum.ConstantVariableTabulated.Variable  wall_geometry=foundation.enum.ConductionWallGeometry.Planar  area=sma_pipe_fa m^2  thickness=1 m  d_in=0.05 m  d_out=0.1 m  L=1 m  th_cond_min=thermal_gate_min_conductivity_W_per_mK W/(K*m)  th_cond=sma_hold_pipe_to_sma_G_W_per_K W/(K*m)  th_cond_TLU=[413, 401, 392, 383, 371, 357, 342] W/(K*m)  temp_TLU=[200, 273, 400, 600, 800, 1000, 1200] K  T_specify=off  T_priority=None  T=0 K  T_nominal_specify=off  T_nominal_value=1  T_nominal_unit=K  Q_specify=off  Q_priority=None  Q=0 W  Q_nominal_specify=off  Q_nominal_value=1  Q_nominal_unit=W
      settings: InternalSimscapePortConfiguration="{\"Bottom\":[],\"Left\":[{\"id\":\"A\",\"label\":\"A\",\"type\":\"foundation.thermal.thermal\"},{\"id\":\"var_th_cond\",\"label\":\"K\",\"type\":\"input\"}],\"Right\":[{\"id\":\"B\",\"label\":\"B\",\"type\":\"foundation.thermal.thermal\"}],\"Top\":[]}"
  SMACooldownNode01HeatFlowPS : nesl_utility/PS-Simulink Converter  PhysicalDomain=network_engine_domain  SubClassName=ps_output  LeftPortType=input  RightPortType=output  PseudoPeriodic=off  Frequencies=[]  VectorFormat=1-D array  Unit=W  AffineConversion=off
  SMACooldownNode01HeatFlowSensor : fl_lib/Thermal/Thermal Sensors/Heat Flow Rate Sensor
  SMACooldownNode02HeatFlowPS : nesl_utility/PS-Simulink Converter  PhysicalDomain=network_engine_domain  SubClassName=ps_output  LeftPortType=input  RightPortType=output  PseudoPeriodic=off  Frequencies=[]  VectorFormat=1-D array  Unit=W  AffineConversion=off
  SMACooldownNode02HeatFlowSensor : fl_lib/Thermal/Thermal Sensors/Heat Flow Rate Sensor
  SMACooldownNode03HeatFlowPS : nesl_utility/PS-Simulink Converter  PhysicalDomain=network_engine_domain  SubClassName=ps_output  LeftPortType=input  RightPortType=output  PseudoPeriodic=off  Frequencies=[]  VectorFormat=1-D array  Unit=W  AffineConversion=off
  SMACooldownNode03HeatFlowSensor : fl_lib/Thermal/Thermal Sensors/Heat Flow Rate Sensor
  SMACooldownNode04HeatFlowPS : nesl_utility/PS-Simulink Converter  PhysicalDomain=network_engine_domain  SubClassName=ps_output  LeftPortType=input  RightPortType=output  PseudoPeriodic=off  Frequencies=[]  VectorFormat=1-D array  Unit=W  AffineConversion=off
  SMACooldownNode04HeatFlowSensor : fl_lib/Thermal/Thermal Sensors/Heat Flow Rate Sensor
  SMACooldownNode05HeatFlowPS : nesl_utility/PS-Simulink Converter  PhysicalDomain=network_engine_domain  SubClassName=ps_output  LeftPortType=input  RightPortType=output  PseudoPeriodic=off  Frequencies=[]  VectorFormat=1-D array  Unit=W  AffineConversion=off
  SMACooldownNode05HeatFlowSensor : fl_lib/Thermal/Thermal Sensors/Heat Flow Rate Sensor
  SMACooldownNode06HeatFlowPS : nesl_utility/PS-Simulink Converter  PhysicalDomain=network_engine_domain  SubClassName=ps_output  LeftPortType=input  RightPortType=output  PseudoPeriodic=off  Frequencies=[]  VectorFormat=1-D array  Unit=W  AffineConversion=off
  SMACooldownNode06HeatFlowSensor : fl_lib/Thermal/Thermal Sensors/Heat Flow Rate Sensor
  SMACooldownNode07HeatFlowPS : nesl_utility/PS-Simulink Converter  PhysicalDomain=network_engine_domain  SubClassName=ps_output  LeftPortType=input  RightPortType=output  PseudoPeriodic=off  Frequencies=[]  VectorFormat=1-D array  Unit=W  AffineConversion=off
  SMACooldownNode07HeatFlowSensor : fl_lib/Thermal/Thermal Sensors/Heat Flow Rate Sensor
  SMACooldownNode08HeatFlowPS : nesl_utility/PS-Simulink Converter  PhysicalDomain=network_engine_domain  SubClassName=ps_output  LeftPortType=input  RightPortType=output  PseudoPeriodic=off  Frequencies=[]  VectorFormat=1-D array  Unit=W  AffineConversion=off
  SMACooldownNode08HeatFlowSensor : fl_lib/Thermal/Thermal Sensors/Heat Flow Rate Sensor
  SMACooldownNode09HeatFlowPS : nesl_utility/PS-Simulink Converter  PhysicalDomain=network_engine_domain  SubClassName=ps_output  LeftPortType=input  RightPortType=output  PseudoPeriodic=off  Frequencies=[]  VectorFormat=1-D array  Unit=W  AffineConversion=off
  SMACooldownNode09HeatFlowSensor : fl_lib/Thermal/Thermal Sensors/Heat Flow Rate Sensor
  SMACooldownNode10HeatFlowPS : nesl_utility/PS-Simulink Converter  PhysicalDomain=network_engine_domain  SubClassName=ps_output  LeftPortType=input  RightPortType=output  PseudoPeriodic=off  Frequencies=[]  VectorFormat=1-D array  Unit=W  AffineConversion=off
  SMACooldownNode10HeatFlowSensor : fl_lib/Thermal/Thermal Sensors/Heat Flow Rate Sensor
  SMACooldownNode11HeatFlowPS : nesl_utility/PS-Simulink Converter  PhysicalDomain=network_engine_domain  SubClassName=ps_output  LeftPortType=input  RightPortType=output  PseudoPeriodic=off  Frequencies=[]  VectorFormat=1-D array  Unit=W  AffineConversion=off
  SMACooldownNode11HeatFlowSensor : fl_lib/Thermal/Thermal Sensors/Heat Flow Rate Sensor
  SMACooldownNode12HeatFlowPS : nesl_utility/PS-Simulink Converter  PhysicalDomain=network_engine_domain  SubClassName=ps_output  LeftPortType=input  RightPortType=output  PseudoPeriodic=off  Frequencies=[]  VectorFormat=1-D array  Unit=W  AffineConversion=off
  SMACooldownNode12HeatFlowSensor : fl_lib/Thermal/Thermal Sensors/Heat Flow Rate Sensor
  SMACooldownNode13HeatFlowPS : nesl_utility/PS-Simulink Converter  PhysicalDomain=network_engine_domain  SubClassName=ps_output  LeftPortType=input  RightPortType=output  PseudoPeriodic=off  Frequencies=[]  VectorFormat=1-D array  Unit=W  AffineConversion=off
  SMACooldownNode13HeatFlowSensor : fl_lib/Thermal/Thermal Sensors/Heat Flow Rate Sensor
  SMACooldownNode14HeatFlowPS : nesl_utility/PS-Simulink Converter  PhysicalDomain=network_engine_domain  SubClassName=ps_output  LeftPortType=input  RightPortType=output  PseudoPeriodic=off  Frequencies=[]  VectorFormat=1-D array  Unit=W  AffineConversion=off
  SMACooldownNode14HeatFlowSensor : fl_lib/Thermal/Thermal Sensors/Heat Flow Rate Sensor
  SMACooldownNode15HeatFlowPS : nesl_utility/PS-Simulink Converter  PhysicalDomain=network_engine_domain  SubClassName=ps_output  LeftPortType=input  RightPortType=output  PseudoPeriodic=off  Frequencies=[]  VectorFormat=1-D array  Unit=W  AffineConversion=off
  SMACooldownNode15HeatFlowSensor : fl_lib/Thermal/Thermal Sensors/Heat Flow Rate Sensor
  SMACooldownNode16HeatFlowPS : nesl_utility/PS-Simulink Converter  PhysicalDomain=network_engine_domain  SubClassName=ps_output  LeftPortType=input  RightPortType=output  PseudoPeriodic=off  Frequencies=[]  VectorFormat=1-D array  Unit=W  AffineConversion=off
  SMACooldownNode16HeatFlowSensor : fl_lib/Thermal/Thermal Sensors/Heat Flow Rate Sensor
  SMACooldownNode17HeatFlowPS : nesl_utility/PS-Simulink Converter  PhysicalDomain=network_engine_domain  SubClassName=ps_output  LeftPortType=input  RightPortType=output  PseudoPeriodic=off  Frequencies=[]  VectorFormat=1-D array  Unit=W  AffineConversion=off
  SMACooldownNode17HeatFlowSensor : fl_lib/Thermal/Thermal Sensors/Heat Flow Rate Sensor
  SMACooldownNode18HeatFlowPS : nesl_utility/PS-Simulink Converter  PhysicalDomain=network_engine_domain  SubClassName=ps_output  LeftPortType=input  RightPortType=output  PseudoPeriodic=off  Frequencies=[]  VectorFormat=1-D array  Unit=W  AffineConversion=off
  SMACooldownNode18HeatFlowSensor : fl_lib/Thermal/Thermal Sensors/Heat Flow Rate Sensor
  SMACooldownNode19HeatFlowPS : nesl_utility/PS-Simulink Converter  PhysicalDomain=network_engine_domain  SubClassName=ps_output  LeftPortType=input  RightPortType=output  PseudoPeriodic=off  Frequencies=[]  VectorFormat=1-D array  Unit=W  AffineConversion=off
  SMACooldownNode19HeatFlowSensor : fl_lib/Thermal/Thermal Sensors/Heat Flow Rate Sensor
  SMACooldownNode20HeatFlowPS : nesl_utility/PS-Simulink Converter  PhysicalDomain=network_engine_domain  SubClassName=ps_output  LeftPortType=input  RightPortType=output  PseudoPeriodic=off  Frequencies=[]  VectorFormat=1-D array  Unit=W  AffineConversion=off
  SMACooldownNode20HeatFlowSensor : fl_lib/Thermal/Thermal Sensors/Heat Flow Rate Sensor
  SMACooldownNode21HeatFlowPS : nesl_utility/PS-Simulink Converter  PhysicalDomain=network_engine_domain  SubClassName=ps_output  LeftPortType=input  RightPortType=output  PseudoPeriodic=off  Frequencies=[]  VectorFormat=1-D array  Unit=W  AffineConversion=off
  SMACooldownNode21HeatFlowSensor : fl_lib/Thermal/Thermal Sensors/Heat Flow Rate Sensor
  SMACooldownPipeNode01FluidTempPS : nesl_utility/PS-Simulink Converter  PhysicalDomain=network_engine_domain  SubClassName=ps_output  LeftPortType=input  RightPortType=output  PseudoPeriodic=off  Frequencies=[]  VectorFormat=1-D array  Unit=K  AffineConversion=off
  SMACooldownPipeNode01FluidTempPressurePS : nesl_utility/PS-Simulink Converter  PhysicalDomain=network_engine_domain  SubClassName=ps_output  LeftPortType=input  RightPortType=output  PseudoPeriodic=off  Frequencies=[]  VectorFormat=1-D array  Unit=MPa  AffineConversion=off
  SMACooldownPipeNode01FluidTempSensor : fl_lib/Thermal Liquid/Sensors/Pressure & Temperature Sensor (TL)  reference=foundation.enum.MeasurementReference.absolute  pressure=true  pressure_spec=foundation.enum.PressureMeasementSpec.Absolute  temperature=true
      settings: InternalSimscapePortConfiguration="{\"Bottom\":[{\"id\":\"T\",\"label\":\"T\",\"type\":\"output\"}],\"Left\":[{\"id\":\"A\",\"label\":\"A\",\"type\":\"foundation.thermal_liquid.thermal_liquid\"}],\"Right\":[{\"id\":\"Pa\",\"label\":\"Pa\",\"type\":\"output\"}],\"Top\":[]}"
  SMACooldownPipeNode11FluidTempPS : nesl_utility/PS-Simulink Converter  PhysicalDomain=network_engine_domain  SubClassName=ps_output  LeftPortType=input  RightPortType=output  PseudoPeriodic=off  Frequencies=[]  VectorFormat=1-D array  Unit=K  AffineConversion=off
  SMACooldownPipeNode11FluidTempPressurePS : nesl_utility/PS-Simulink Converter  PhysicalDomain=network_engine_domain  SubClassName=ps_output  LeftPortType=input  RightPortType=output  PseudoPeriodic=off  Frequencies=[]  VectorFormat=1-D array  Unit=MPa  AffineConversion=off
  SMACooldownPipeNode11FluidTempSensor : fl_lib/Thermal Liquid/Sensors/Pressure & Temperature Sensor (TL)  reference=foundation.enum.MeasurementReference.absolute  pressure=true  pressure_spec=foundation.enum.PressureMeasementSpec.Absolute  temperature=true
      settings: InternalSimscapePortConfiguration="{\"Bottom\":[{\"id\":\"T\",\"label\":\"T\",\"type\":\"output\"}],\"Left\":[{\"id\":\"A\",\"label\":\"A\",\"type\":\"foundation.thermal_liquid.thermal_liquid\"}],\"Right\":[{\"id\":\"Pa\",\"label\":\"Pa\",\"type\":\"output\"}],\"Top\":[]}"
  SMACooldownPipeNode21FluidTempPS : nesl_utility/PS-Simulink Converter  PhysicalDomain=network_engine_domain  SubClassName=ps_output  LeftPortType=input  RightPortType=output  PseudoPeriodic=off  Frequencies=[]  VectorFormat=1-D array  Unit=K  AffineConversion=off
  SMACooldownPipeNode21FluidTempPressurePS : nesl_utility/PS-Simulink Converter  PhysicalDomain=network_engine_domain  SubClassName=ps_output  LeftPortType=input  RightPortType=output  PseudoPeriodic=off  Frequencies=[]  VectorFormat=1-D array  Unit=MPa  AffineConversion=off
  SMACooldownPipeNode21FluidTempSensor : fl_lib/Thermal Liquid/Sensors/Pressure & Temperature Sensor (TL)  reference=foundation.enum.MeasurementReference.absolute  pressure=true  pressure_spec=foundation.enum.PressureMeasementSpec.Absolute  temperature=true
      settings: InternalSimscapePortConfiguration="{\"Bottom\":[{\"id\":\"T\",\"label\":\"T\",\"type\":\"output\"}],\"Left\":[{\"id\":\"A\",\"label\":\"A\",\"type\":\"foundation.thermal_liquid.thermal_liquid\"}],\"Right\":[{\"id\":\"Pa\",\"label\":\"Pa\",\"type\":\"output\"}],\"Top\":[]}"
  SMAHoldNode01HeatFlowPS : nesl_utility/PS-Simulink Converter  PhysicalDomain=network_engine_domain  SubClassName=ps_output  LeftPortType=input  RightPortType=output  PseudoPeriodic=off  Frequencies=[]  VectorFormat=1-D array  Unit=W  AffineConversion=off
  SMAHoldNode01HeatFlowSensor : fl_lib/Thermal/Thermal Sensors/Heat Flow Rate Sensor
  SMAHoldNode02HeatFlowPS : nesl_utility/PS-Simulink Converter  PhysicalDomain=network_engine_domain  SubClassName=ps_output  LeftPortType=input  RightPortType=output  PseudoPeriodic=off  Frequencies=[]  VectorFormat=1-D array  Unit=W  AffineConversion=off
  SMAHoldNode02HeatFlowSensor : fl_lib/Thermal/Thermal Sensors/Heat Flow Rate Sensor
  SMAHoldNode03HeatFlowPS : nesl_utility/PS-Simulink Converter  PhysicalDomain=network_engine_domain  SubClassName=ps_output  LeftPortType=input  RightPortType=output  PseudoPeriodic=off  Frequencies=[]  VectorFormat=1-D array  Unit=W  AffineConversion=off
  SMAHoldNode03HeatFlowSensor : fl_lib/Thermal/Thermal Sensors/Heat Flow Rate Sensor
  SMAHoldNode04HeatFlowPS : nesl_utility/PS-Simulink Converter  PhysicalDomain=network_engine_domain  SubClassName=ps_output  LeftPortType=input  RightPortType=output  PseudoPeriodic=off  Frequencies=[]  VectorFormat=1-D array  Unit=W  AffineConversion=off
  SMAHoldNode04HeatFlowSensor : fl_lib/Thermal/Thermal Sensors/Heat Flow Rate Sensor
  SMAHoldNode05HeatFlowPS : nesl_utility/PS-Simulink Converter  PhysicalDomain=network_engine_domain  SubClassName=ps_output  LeftPortType=input  RightPortType=output  PseudoPeriodic=off  Frequencies=[]  VectorFormat=1-D array  Unit=W  AffineConversion=off
  SMAHoldNode05HeatFlowSensor : fl_lib/Thermal/Thermal Sensors/Heat Flow Rate Sensor
  SMAHoldNode06HeatFlowPS : nesl_utility/PS-Simulink Converter  PhysicalDomain=network_engine_domain  SubClassName=ps_output  LeftPortType=input  RightPortType=output  PseudoPeriodic=off  Frequencies=[]  VectorFormat=1-D array  Unit=W  AffineConversion=off
  SMAHoldNode06HeatFlowSensor : fl_lib/Thermal/Thermal Sensors/Heat Flow Rate Sensor
  SMAHoldNode07HeatFlowPS : nesl_utility/PS-Simulink Converter  PhysicalDomain=network_engine_domain  SubClassName=ps_output  LeftPortType=input  RightPortType=output  PseudoPeriodic=off  Frequencies=[]  VectorFormat=1-D array  Unit=W  AffineConversion=off
  SMAHoldNode07HeatFlowSensor : fl_lib/Thermal/Thermal Sensors/Heat Flow Rate Sensor
  SMAHoldNode08HeatFlowPS : nesl_utility/PS-Simulink Converter  PhysicalDomain=network_engine_domain  SubClassName=ps_output  LeftPortType=input  RightPortType=output  PseudoPeriodic=off  Frequencies=[]  VectorFormat=1-D array  Unit=W  AffineConversion=off
  SMAHoldNode08HeatFlowSensor : fl_lib/Thermal/Thermal Sensors/Heat Flow Rate Sensor
  SMAHoldNode09HeatFlowPS : nesl_utility/PS-Simulink Converter  PhysicalDomain=network_engine_domain  SubClassName=ps_output  LeftPortType=input  RightPortType=output  PseudoPeriodic=off  Frequencies=[]  VectorFormat=1-D array  Unit=W  AffineConversion=off
  SMAHoldNode09HeatFlowSensor : fl_lib/Thermal/Thermal Sensors/Heat Flow Rate Sensor
  SMAHoldNode10HeatFlowPS : nesl_utility/PS-Simulink Converter  PhysicalDomain=network_engine_domain  SubClassName=ps_output  LeftPortType=input  RightPortType=output  PseudoPeriodic=off  Frequencies=[]  VectorFormat=1-D array  Unit=W  AffineConversion=off
  SMAHoldNode10HeatFlowSensor : fl_lib/Thermal/Thermal Sensors/Heat Flow Rate Sensor
  SMAHoldNode11HeatFlowPS : nesl_utility/PS-Simulink Converter  PhysicalDomain=network_engine_domain  SubClassName=ps_output  LeftPortType=input  RightPortType=output  PseudoPeriodic=off  Frequencies=[]  VectorFormat=1-D array  Unit=W  AffineConversion=off
  SMAHoldNode11HeatFlowSensor : fl_lib/Thermal/Thermal Sensors/Heat Flow Rate Sensor
  SMAHoldNode12HeatFlowPS : nesl_utility/PS-Simulink Converter  PhysicalDomain=network_engine_domain  SubClassName=ps_output  LeftPortType=input  RightPortType=output  PseudoPeriodic=off  Frequencies=[]  VectorFormat=1-D array  Unit=W  AffineConversion=off
  SMAHoldNode12HeatFlowSensor : fl_lib/Thermal/Thermal Sensors/Heat Flow Rate Sensor
  SMAHoldNode13HeatFlowPS : nesl_utility/PS-Simulink Converter  PhysicalDomain=network_engine_domain  SubClassName=ps_output  LeftPortType=input  RightPortType=output  PseudoPeriodic=off  Frequencies=[]  VectorFormat=1-D array  Unit=W  AffineConversion=off
  SMAHoldNode13HeatFlowSensor : fl_lib/Thermal/Thermal Sensors/Heat Flow Rate Sensor
  SMAHoldNode14HeatFlowPS : nesl_utility/PS-Simulink Converter  PhysicalDomain=network_engine_domain  SubClassName=ps_output  LeftPortType=input  RightPortType=output  PseudoPeriodic=off  Frequencies=[]  VectorFormat=1-D array  Unit=W  AffineConversion=off
  SMAHoldNode14HeatFlowSensor : fl_lib/Thermal/Thermal Sensors/Heat Flow Rate Sensor
  SMAHoldNode15HeatFlowPS : nesl_utility/PS-Simulink Converter  PhysicalDomain=network_engine_domain  SubClassName=ps_output  LeftPortType=input  RightPortType=output  PseudoPeriodic=off  Frequencies=[]  VectorFormat=1-D array  Unit=W  AffineConversion=off
  SMAHoldNode15HeatFlowSensor : fl_lib/Thermal/Thermal Sensors/Heat Flow Rate Sensor
  SMAHoldNode16HeatFlowPS : nesl_utility/PS-Simulink Converter  PhysicalDomain=network_engine_domain  SubClassName=ps_output  LeftPortType=input  RightPortType=output  PseudoPeriodic=off  Frequencies=[]  VectorFormat=1-D array  Unit=W  AffineConversion=off
  SMAHoldNode16HeatFlowSensor : fl_lib/Thermal/Thermal Sensors/Heat Flow Rate Sensor
  SMAHoldNode17HeatFlowPS : nesl_utility/PS-Simulink Converter  PhysicalDomain=network_engine_domain  SubClassName=ps_output  LeftPortType=input  RightPortType=output  PseudoPeriodic=off  Frequencies=[]  VectorFormat=1-D array  Unit=W  AffineConversion=off
  SMAHoldNode17HeatFlowSensor : fl_lib/Thermal/Thermal Sensors/Heat Flow Rate Sensor
  SMAHoldNode18HeatFlowPS : nesl_utility/PS-Simulink Converter  PhysicalDomain=network_engine_domain  SubClassName=ps_output  LeftPortType=input  RightPortType=output  PseudoPeriodic=off  Frequencies=[]  VectorFormat=1-D array  Unit=W  AffineConversion=off
  SMAHoldNode18HeatFlowSensor : fl_lib/Thermal/Thermal Sensors/Heat Flow Rate Sensor
  SMAHoldNode19HeatFlowPS : nesl_utility/PS-Simulink Converter  PhysicalDomain=network_engine_domain  SubClassName=ps_output  LeftPortType=input  RightPortType=output  PseudoPeriodic=off  Frequencies=[]  VectorFormat=1-D array  Unit=W  AffineConversion=off
  SMAHoldNode19HeatFlowSensor : fl_lib/Thermal/Thermal Sensors/Heat Flow Rate Sensor
  SMAHoldNode20HeatFlowPS : nesl_utility/PS-Simulink Converter  PhysicalDomain=network_engine_domain  SubClassName=ps_output  LeftPortType=input  RightPortType=output  PseudoPeriodic=off  Frequencies=[]  VectorFormat=1-D array  Unit=W  AffineConversion=off
  SMAHoldNode20HeatFlowSensor : fl_lib/Thermal/Thermal Sensors/Heat Flow Rate Sensor
  SMAHoldNode21HeatFlowPS : nesl_utility/PS-Simulink Converter  PhysicalDomain=network_engine_domain  SubClassName=ps_output  LeftPortType=input  RightPortType=output  PseudoPeriodic=off  Frequencies=[]  VectorFormat=1-D array  Unit=W  AffineConversion=off
  SMAHoldNode21HeatFlowSensor : fl_lib/Thermal/Thermal Sensors/Heat Flow Rate Sensor
  SMAHoldPipeNode01FluidTempPS : nesl_utility/PS-Simulink Converter  PhysicalDomain=network_engine_domain  SubClassName=ps_output  LeftPortType=input  RightPortType=output  PseudoPeriodic=off  Frequencies=[]  VectorFormat=1-D array  Unit=K  AffineConversion=off
  SMAHoldPipeNode01FluidTempPressurePS : nesl_utility/PS-Simulink Converter  PhysicalDomain=network_engine_domain  SubClassName=ps_output  LeftPortType=input  RightPortType=output  PseudoPeriodic=off  Frequencies=[]  VectorFormat=1-D array  Unit=MPa  AffineConversion=off
  SMAHoldPipeNode01FluidTempSensor : fl_lib/Thermal Liquid/Sensors/Pressure & Temperature Sensor (TL)  reference=foundation.enum.MeasurementReference.absolute  pressure=true  pressure_spec=foundation.enum.PressureMeasementSpec.Absolute  temperature=true
      settings: InternalSimscapePortConfiguration="{\"Bottom\":[{\"id\":\"T\",\"label\":\"T\",\"type\":\"output\"}],\"Left\":[{\"id\":\"A\",\"label\":\"A\",\"type\":\"foundation.thermal_liquid.thermal_liquid\"}],\"Right\":[{\"id\":\"Pa\",\"label\":\"Pa\",\"type\":\"output\"}],\"Top\":[]}"
  SMAHoldPipeNode11FluidTempPS : nesl_utility/PS-Simulink Converter  PhysicalDomain=network_engine_domain  SubClassName=ps_output  LeftPortType=input  RightPortType=output  PseudoPeriodic=off  Frequencies=[]  VectorFormat=1-D array  Unit=K  AffineConversion=off
  SMAHoldPipeNode11FluidTempPressurePS : nesl_utility/PS-Simulink Converter  PhysicalDomain=network_engine_domain  SubClassName=ps_output  LeftPortType=input  RightPortType=output  PseudoPeriodic=off  Frequencies=[]  VectorFormat=1-D array  Unit=MPa  AffineConversion=off
  SMAHoldPipeNode11FluidTempSensor : fl_lib/Thermal Liquid/Sensors/Pressure & Temperature Sensor (TL)  reference=foundation.enum.MeasurementReference.absolute  pressure=true  pressure_spec=foundation.enum.PressureMeasementSpec.Absolute  temperature=true
      settings: InternalSimscapePortConfiguration="{\"Bottom\":[{\"id\":\"T\",\"label\":\"T\",\"type\":\"output\"}],\"Left\":[{\"id\":\"A\",\"label\":\"A\",\"type\":\"foundation.thermal_liquid.thermal_liquid\"}],\"Right\":[{\"id\":\"Pa\",\"label\":\"Pa\",\"type\":\"output\"}],\"Top\":[]}"
  SMAHoldPipeNode21FluidTempPS : nesl_utility/PS-Simulink Converter  PhysicalDomain=network_engine_domain  SubClassName=ps_output  LeftPortType=input  RightPortType=output  PseudoPeriodic=off  Frequencies=[]  VectorFormat=1-D array  Unit=K  AffineConversion=off
  SMAHoldPipeNode21FluidTempPressurePS : nesl_utility/PS-Simulink Converter  PhysicalDomain=network_engine_domain  SubClassName=ps_output  LeftPortType=input  RightPortType=output  PseudoPeriodic=off  Frequencies=[]  VectorFormat=1-D array  Unit=MPa  AffineConversion=off
  SMAHoldPipeNode21FluidTempSensor : fl_lib/Thermal Liquid/Sensors/Pressure & Temperature Sensor (TL)  reference=foundation.enum.MeasurementReference.absolute  pressure=true  pressure_spec=foundation.enum.PressureMeasementSpec.Absolute  temperature=true
      settings: InternalSimscapePortConfiguration="{\"Bottom\":[{\"id\":\"T\",\"label\":\"T\",\"type\":\"output\"}],\"Left\":[{\"id\":\"A\",\"label\":\"A\",\"type\":\"foundation.thermal_liquid.thermal_liquid\"}],\"Right\":[{\"id\":\"Pa\",\"label\":\"Pa\",\"type\":\"output\"}],\"Top\":[]}"
  Subsystem2 : Subsystem
  ToWorkspace_sma_cooldown_node01_heatflow_W : ToWorkspace  VariableName=sma_cooldown_node01_heatflow_W  SaveFormat=Structure With Time  SampleTime=-1
  ToWorkspace_sma_cooldown_node02_heatflow_W : ToWorkspace  VariableName=sma_cooldown_node02_heatflow_W  SaveFormat=Structure With Time  SampleTime=-1
  ToWorkspace_sma_cooldown_node03_heatflow_W : ToWorkspace  VariableName=sma_cooldown_node03_heatflow_W  SaveFormat=Structure With Time  SampleTime=-1
  ToWorkspace_sma_cooldown_node04_heatflow_W : ToWorkspace  VariableName=sma_cooldown_node04_heatflow_W  SaveFormat=Structure With Time  SampleTime=-1
  ToWorkspace_sma_cooldown_node05_heatflow_W : ToWorkspace  VariableName=sma_cooldown_node05_heatflow_W  SaveFormat=Structure With Time  SampleTime=-1
  ToWorkspace_sma_cooldown_node06_heatflow_W : ToWorkspace  VariableName=sma_cooldown_node06_heatflow_W  SaveFormat=Structure With Time  SampleTime=-1
  ToWorkspace_sma_cooldown_node07_heatflow_W : ToWorkspace  VariableName=sma_cooldown_node07_heatflow_W  SaveFormat=Structure With Time  SampleTime=-1
  ToWorkspace_sma_cooldown_node08_heatflow_W : ToWorkspace  VariableName=sma_cooldown_node08_heatflow_W  SaveFormat=Structure With Time  SampleTime=-1
  ToWorkspace_sma_cooldown_node09_heatflow_W : ToWorkspace  VariableName=sma_cooldown_node09_heatflow_W  SaveFormat=Structure With Time  SampleTime=-1
  ToWorkspace_sma_cooldown_node10_heatflow_W : ToWorkspace  VariableName=sma_cooldown_node10_heatflow_W  SaveFormat=Structure With Time  SampleTime=-1
  ToWorkspace_sma_cooldown_node11_heatflow_W : ToWorkspace  VariableName=sma_cooldown_node11_heatflow_W  SaveFormat=Structure With Time  SampleTime=-1
  ToWorkspace_sma_cooldown_node12_heatflow_W : ToWorkspace  VariableName=sma_cooldown_node12_heatflow_W  SaveFormat=Structure With Time  SampleTime=-1
  ToWorkspace_sma_cooldown_node13_heatflow_W : ToWorkspace  VariableName=sma_cooldown_node13_heatflow_W  SaveFormat=Structure With Time  SampleTime=-1
  ToWorkspace_sma_cooldown_node14_heatflow_W : ToWorkspace  VariableName=sma_cooldown_node14_heatflow_W  SaveFormat=Structure With Time  SampleTime=-1
  ToWorkspace_sma_cooldown_node15_heatflow_W : ToWorkspace  VariableName=sma_cooldown_node15_heatflow_W  SaveFormat=Structure With Time  SampleTime=-1
  ToWorkspace_sma_cooldown_node16_heatflow_W : ToWorkspace  VariableName=sma_cooldown_node16_heatflow_W  SaveFormat=Structure With Time  SampleTime=-1
  ToWorkspace_sma_cooldown_node17_heatflow_W : ToWorkspace  VariableName=sma_cooldown_node17_heatflow_W  SaveFormat=Structure With Time  SampleTime=-1
  ToWorkspace_sma_cooldown_node18_heatflow_W : ToWorkspace  VariableName=sma_cooldown_node18_heatflow_W  SaveFormat=Structure With Time  SampleTime=-1
  ToWorkspace_sma_cooldown_node19_heatflow_W : ToWorkspace  VariableName=sma_cooldown_node19_heatflow_W  SaveFormat=Structure With Time  SampleTime=-1
  ToWorkspace_sma_cooldown_node20_heatflow_W : ToWorkspace  VariableName=sma_cooldown_node20_heatflow_W  SaveFormat=Structure With Time  SampleTime=-1
  ToWorkspace_sma_cooldown_node21_heatflow_W : ToWorkspace  VariableName=sma_cooldown_node21_heatflow_W  SaveFormat=Structure With Time  SampleTime=-1
  ToWorkspace_sma_cooldown_pipe_node01_fluid_temp_out : ToWorkspace  VariableName=sma_cooldown_pipe_node01_fluid_temp_out  SaveFormat=Structure With Time  SampleTime=-1
  ToWorkspace_sma_cooldown_pipe_node01_pressure_MPa : ToWorkspace  VariableName=sma_cooldown_pipe_node01_pressure_MPa  SaveFormat=Structure With Time  SampleTime=-1
  ToWorkspace_sma_cooldown_pipe_node11_fluid_temp_out : ToWorkspace  VariableName=sma_cooldown_pipe_node11_fluid_temp_out  SaveFormat=Structure With Time  SampleTime=-1
  ToWorkspace_sma_cooldown_pipe_node11_pressure_MPa : ToWorkspace  VariableName=sma_cooldown_pipe_node11_pressure_MPa  SaveFormat=Structure With Time  SampleTime=-1
  ToWorkspace_sma_cooldown_pipe_node21_fluid_temp_out : ToWorkspace  VariableName=sma_cooldown_pipe_node21_fluid_temp_out  SaveFormat=Structure With Time  SampleTime=-1
  ToWorkspace_sma_cooldown_pipe_node21_pressure_MPa : ToWorkspace  VariableName=sma_cooldown_pipe_node21_pressure_MPa  SaveFormat=Structure With Time  SampleTime=-1
  ToWorkspace_sma_hold_node01_heatflow_W : ToWorkspace  VariableName=sma_hold_node01_heatflow_W  SaveFormat=Structure With Time  SampleTime=-1
  ToWorkspace_sma_hold_node02_heatflow_W : ToWorkspace  VariableName=sma_hold_node02_heatflow_W  SaveFormat=Structure With Time  SampleTime=-1
  ToWorkspace_sma_hold_node03_heatflow_W : ToWorkspace  VariableName=sma_hold_node03_heatflow_W  SaveFormat=Structure With Time  SampleTime=-1
  ToWorkspace_sma_hold_node04_heatflow_W : ToWorkspace  VariableName=sma_hold_node04_heatflow_W  SaveFormat=Structure With Time  SampleTime=-1
  ToWorkspace_sma_hold_node05_heatflow_W : ToWorkspace  VariableName=sma_hold_node05_heatflow_W  SaveFormat=Structure With Time  SampleTime=-1
  ToWorkspace_sma_hold_node06_heatflow_W : ToWorkspace  VariableName=sma_hold_node06_heatflow_W  SaveFormat=Structure With Time  SampleTime=-1
  ToWorkspace_sma_hold_node07_heatflow_W : ToWorkspace  VariableName=sma_hold_node07_heatflow_W  SaveFormat=Structure With Time  SampleTime=-1
  ToWorkspace_sma_hold_node08_heatflow_W : ToWorkspace  VariableName=sma_hold_node08_heatflow_W  SaveFormat=Structure With Time  SampleTime=-1
  ToWorkspace_sma_hold_node09_heatflow_W : ToWorkspace  VariableName=sma_hold_node09_heatflow_W  SaveFormat=Structure With Time  SampleTime=-1
  ToWorkspace_sma_hold_node10_heatflow_W : ToWorkspace  VariableName=sma_hold_node10_heatflow_W  SaveFormat=Structure With Time  SampleTime=-1
  ToWorkspace_sma_hold_node11_heatflow_W : ToWorkspace  VariableName=sma_hold_node11_heatflow_W  SaveFormat=Structure With Time  SampleTime=-1
  ToWorkspace_sma_hold_node12_heatflow_W : ToWorkspace  VariableName=sma_hold_node12_heatflow_W  SaveFormat=Structure With Time  SampleTime=-1
  ToWorkspace_sma_hold_node13_heatflow_W : ToWorkspace  VariableName=sma_hold_node13_heatflow_W  SaveFormat=Structure With Time  SampleTime=-1
  ToWorkspace_sma_hold_node14_heatflow_W : ToWorkspace  VariableName=sma_hold_node14_heatflow_W  SaveFormat=Structure With Time  SampleTime=-1
  ToWorkspace_sma_hold_node15_heatflow_W : ToWorkspace  VariableName=sma_hold_node15_heatflow_W  SaveFormat=Structure With Time  SampleTime=-1
  ToWorkspace_sma_hold_node16_heatflow_W : ToWorkspace  VariableName=sma_hold_node16_heatflow_W  SaveFormat=Structure With Time  SampleTime=-1
  ToWorkspace_sma_hold_node17_heatflow_W : ToWorkspace  VariableName=sma_hold_node17_heatflow_W  SaveFormat=Structure With Time  SampleTime=-1
  ToWorkspace_sma_hold_node18_heatflow_W : ToWorkspace  VariableName=sma_hold_node18_heatflow_W  SaveFormat=Structure With Time  SampleTime=-1
  ToWorkspace_sma_hold_node19_heatflow_W : ToWorkspace  VariableName=sma_hold_node19_heatflow_W  SaveFormat=Structure With Time  SampleTime=-1
  ToWorkspace_sma_hold_node20_heatflow_W : ToWorkspace  VariableName=sma_hold_node20_heatflow_W  SaveFormat=Structure With Time  SampleTime=-1
  ToWorkspace_sma_hold_node21_heatflow_W : ToWorkspace  VariableName=sma_hold_node21_heatflow_W  SaveFormat=Structure With Time  SampleTime=-1
  ToWorkspace_sma_hold_pipe_node01_fluid_temp_out : ToWorkspace  VariableName=sma_hold_pipe_node01_fluid_temp_out  SaveFormat=Structure With Time  SampleTime=-1
  ToWorkspace_sma_hold_pipe_node01_pressure_MPa : ToWorkspace  VariableName=sma_hold_pipe_node01_pressure_MPa  SaveFormat=Structure With Time  SampleTime=-1
  ToWorkspace_sma_hold_pipe_node11_fluid_temp_out : ToWorkspace  VariableName=sma_hold_pipe_node11_fluid_temp_out  SaveFormat=Structure With Time  SampleTime=-1
  ToWorkspace_sma_hold_pipe_node11_pressure_MPa : ToWorkspace  VariableName=sma_hold_pipe_node11_pressure_MPa  SaveFormat=Structure With Time  SampleTime=-1
  ToWorkspace_sma_hold_pipe_node21_fluid_temp_out : ToWorkspace  VariableName=sma_hold_pipe_node21_fluid_temp_out  SaveFormat=Structure With Time  SampleTime=-1
  ToWorkspace_sma_hold_pipe_node21_pressure_MPa : ToWorkspace  VariableName=sma_hold_pipe_node21_pressure_MPa  SaveFormat=Structure With Time  SampleTime=-1
  Conn1 : PMIOPort  Side=Left
  Conn2 : PMIOPort  Port=2  Side=Left
  Conn3 : PMIOPort  Port=3  Side=Left
  Conn4 : PMIOPort  Port=4  Side=Left
  NodeTemp21Out : Outport
  wires:
  ConstitutiveHeat21_W/1 -> Subsystem2/1(ConstitutiveHeat21_W)
  Subsystem2/1(NodeTemp21Out) -> NodeTemp21Out/1
  HoldThermalGateCommandFromWorkspace/1 -> HoldThermalGateCommandPS/1
  CooldownThermalGateCommandFromWorkspace/1 -> CooldownThermalGateCommandPS/1
  SMAHoldPipeNode01FluidTempPS/1 -> ToWorkspace_sma_hold_pipe_node01_fluid_temp_out/1
  SMAHoldPipeNode01FluidTempPressurePS/1 -> ToWorkspace_sma_hold_pipe_node01_pressure_MPa/1
  SMAHoldPipeNode11FluidTempPS/1 -> ToWorkspace_sma_hold_pipe_node11_fluid_temp_out/1
  SMAHoldPipeNode11FluidTempPressurePS/1 -> ToWorkspace_sma_hold_pipe_node11_pressure_MPa/1
  SMAHoldPipeNode21FluidTempPS/1 -> ToWorkspace_sma_hold_pipe_node21_fluid_temp_out/1
  SMAHoldPipeNode21FluidTempPressurePS/1 -> ToWorkspace_sma_hold_pipe_node21_pressure_MPa/1
  SMACooldownPipeNode01FluidTempPS/1 -> ToWorkspace_sma_cooldown_pipe_node01_fluid_temp_out/1
  SMACooldownPipeNode01FluidTempPressurePS/1 -> ToWorkspace_sma_cooldown_pipe_node01_pressure_MPa/1
  SMACooldownPipeNode11FluidTempPS/1 -> ToWorkspace_sma_cooldown_pipe_node11_fluid_temp_out/1
  SMACooldownPipeNode11FluidTempPressurePS/1 -> ToWorkspace_sma_cooldown_pipe_node11_pressure_MPa/1
  SMACooldownPipeNode21FluidTempPS/1 -> ToWorkspace_sma_cooldown_pipe_node21_fluid_temp_out/1
  SMACooldownPipeNode21FluidTempPressurePS/1 -> ToWorkspace_sma_cooldown_pipe_node21_pressure_MPa/1
  SMAHoldNode01HeatFlowPS/1 -> ToWorkspace_sma_hold_node01_heatflow_W/1
  SMAHoldNode02HeatFlowPS/1 -> ToWorkspace_sma_hold_node02_heatflow_W/1
  SMAHoldNode03HeatFlowPS/1 -> ToWorkspace_sma_hold_node03_heatflow_W/1
  SMAHoldNode04HeatFlowPS/1 -> ToWorkspace_sma_hold_node04_heatflow_W/1
  SMAHoldNode05HeatFlowPS/1 -> ToWorkspace_sma_hold_node05_heatflow_W/1
  SMAHoldNode06HeatFlowPS/1 -> ToWorkspace_sma_hold_node06_heatflow_W/1
  SMAHoldNode07HeatFlowPS/1 -> ToWorkspace_sma_hold_node07_heatflow_W/1
  SMAHoldNode08HeatFlowPS/1 -> ToWorkspace_sma_hold_node08_heatflow_W/1
  SMAHoldNode09HeatFlowPS/1 -> ToWorkspace_sma_hold_node09_heatflow_W/1
  SMAHoldNode10HeatFlowPS/1 -> ToWorkspace_sma_hold_node10_heatflow_W/1
  SMAHoldNode11HeatFlowPS/1 -> ToWorkspace_sma_hold_node11_heatflow_W/1
  SMAHoldNode12HeatFlowPS/1 -> ToWorkspace_sma_hold_node12_heatflow_W/1
  SMAHoldNode13HeatFlowPS/1 -> ToWorkspace_sma_hold_node13_heatflow_W/1
  SMAHoldNode14HeatFlowPS/1 -> ToWorkspace_sma_hold_node14_heatflow_W/1
  SMAHoldNode15HeatFlowPS/1 -> ToWorkspace_sma_hold_node15_heatflow_W/1
  SMAHoldNode16HeatFlowPS/1 -> ToWorkspace_sma_hold_node16_heatflow_W/1
  SMAHoldNode17HeatFlowPS/1 -> ToWorkspace_sma_hold_node17_heatflow_W/1
  SMAHoldNode18HeatFlowPS/1 -> ToWorkspace_sma_hold_node18_heatflow_W/1
  SMAHoldNode19HeatFlowPS/1 -> ToWorkspace_sma_hold_node19_heatflow_W/1
  SMAHoldNode20HeatFlowPS/1 -> ToWorkspace_sma_hold_node20_heatflow_W/1
  SMAHoldNode21HeatFlowPS/1 -> ToWorkspace_sma_hold_node21_heatflow_W/1
  SMACooldownNode01HeatFlowPS/1 -> ToWorkspace_sma_cooldown_node01_heatflow_W/1
  SMACooldownNode02HeatFlowPS/1 -> ToWorkspace_sma_cooldown_node02_heatflow_W/1
  SMACooldownNode03HeatFlowPS/1 -> ToWorkspace_sma_cooldown_node03_heatflow_W/1
  SMACooldownNode04HeatFlowPS/1 -> ToWorkspace_sma_cooldown_node04_heatflow_W/1
  SMACooldownNode05HeatFlowPS/1 -> ToWorkspace_sma_cooldown_node05_heatflow_W/1
  SMACooldownNode06HeatFlowPS/1 -> ToWorkspace_sma_cooldown_node06_heatflow_W/1
  SMACooldownNode07HeatFlowPS/1 -> ToWorkspace_sma_cooldown_node07_heatflow_W/1
  SMACooldownNode08HeatFlowPS/1 -> ToWorkspace_sma_cooldown_node08_heatflow_W/1
  SMACooldownNode09HeatFlowPS/1 -> ToWorkspace_sma_cooldown_node09_heatflow_W/1
  SMACooldownNode10HeatFlowPS/1 -> ToWorkspace_sma_cooldown_node10_heatflow_W/1
  SMACooldownNode11HeatFlowPS/1 -> ToWorkspace_sma_cooldown_node11_heatflow_W/1
  SMACooldownNode12HeatFlowPS/1 -> ToWorkspace_sma_cooldown_node12_heatflow_W/1
  SMACooldownNode13HeatFlowPS/1 -> ToWorkspace_sma_cooldown_node13_heatflow_W/1
  SMACooldownNode14HeatFlowPS/1 -> ToWorkspace_sma_cooldown_node14_heatflow_W/1
  SMACooldownNode15HeatFlowPS/1 -> ToWorkspace_sma_cooldown_node15_heatflow_W/1
  SMACooldownNode16HeatFlowPS/1 -> ToWorkspace_sma_cooldown_node16_heatflow_W/1
  SMACooldownNode17HeatFlowPS/1 -> ToWorkspace_sma_cooldown_node17_heatflow_W/1
  SMACooldownNode18HeatFlowPS/1 -> ToWorkspace_sma_cooldown_node18_heatflow_W/1
  SMACooldownNode19HeatFlowPS/1 -> ToWorkspace_sma_cooldown_node19_heatflow_W/1
  SMACooldownNode20HeatFlowPS/1 -> ToWorkspace_sma_cooldown_node20_heatflow_W/1
  SMACooldownNode21HeatFlowPS/1 -> ToWorkspace_sma_cooldown_node21_heatflow_W/1
  connections:
  CooldownPipe_020/LConn1 -- CooldownPipe_021/RConn1
  CooldownPipe_019/LConn1 -- CooldownPipe_020/RConn1
  CooldownPipe_018/LConn1 -- CooldownPipe_019/RConn1
  CooldownPipe_017/LConn1 -- CooldownPipe_018/RConn1
  CooldownPipe_016/LConn1 -- CooldownPipe_017/RConn1
  CooldownPipe_015/LConn1 -- CooldownPipe_016/RConn1
  CooldownPipe_014/LConn1 -- CooldownPipe_015/RConn1
  CooldownPipe_013/LConn1 -- CooldownPipe_014/RConn1
  CooldownPipe_012/LConn1 -- CooldownPipe_013/RConn1
  CooldownPipe_010/LConn1 -- CooldownPipe_011/RConn1
  CooldownPipe_009/LConn1 -- CooldownPipe_010/RConn1
  CooldownPipe_008/LConn1 -- CooldownPipe_009/RConn1
  CooldownPipe_007/LConn1 -- CooldownPipe_008/RConn1
  CooldownPipe_006/LConn1 -- CooldownPipe_007/RConn1
  CooldownPipe_005/LConn1 -- CooldownPipe_006/RConn1
  CooldownPipe_004/LConn1 -- CooldownPipe_005/RConn1
  CooldownPipe_003/LConn1 -- CooldownPipe_004/RConn1
  CooldownPipe_002/LConn1 -- CooldownPipe_003/RConn1
  CooldownPipe_001/LConn1 -- CooldownPipe_002/RConn1
  HoldPipe_002/LConn1 -- HoldPipe_001/RConn1
  HoldPipe_003/LConn1 -- HoldPipe_002/RConn1
  HoldPipe_004/LConn1 -- HoldPipe_003/RConn1
  HoldPipe_005/LConn1 -- HoldPipe_004/RConn1
  HoldPipe_006/LConn1 -- HoldPipe_005/RConn1
  HoldPipe_007/LConn1 -- HoldPipe_006/RConn1
  HoldPipe_008/LConn1 -- HoldPipe_007/RConn1
  HoldPipe_009/LConn1 -- HoldPipe_008/RConn1
  HoldPipe_010/LConn1 -- HoldPipe_009/RConn1
  HoldPipe_012/LConn1 -- HoldPipe_011/RConn1
  HoldPipe_013/LConn1 -- HoldPipe_012/RConn1
  HoldPipe_014/LConn1 -- HoldPipe_013/RConn1
  HoldPipe_015/LConn1 -- HoldPipe_014/RConn1
  HoldPipe_016/LConn1 -- HoldPipe_015/RConn1
  HoldPipe_017/LConn1 -- HoldPipe_016/RConn1
  HoldPipe_018/LConn1 -- HoldPipe_017/RConn1
  HoldPipe_019/LConn1 -- HoldPipe_018/RConn1
  HoldPipe_020/LConn1 -- HoldPipe_019/RConn1
  HoldPipe_021/LConn1 -- HoldPipe_020/RConn1
  Conn1/RConn1 -- HoldPipe_021/RConn1 -- SMAHoldPipeNode21FluidTempSensor/LConn1
  CooldownPipe_021/LConn2 -- CooldownThermalGate_021/LConn1
  HoldPipe_021/LConn2 -- HoldThermalGate_021/LConn1
  CooldownPipe_020/LConn2 -- CooldownThermalGate_020/LConn1
  HoldPipe_020/LConn2 -- HoldThermalGate_020/LConn1
  CooldownPipe_019/LConn2 -- CooldownThermalGate_019/LConn1
  HoldPipe_019/LConn2 -- HoldThermalGate_019/LConn1
  CooldownPipe_018/LConn2 -- CooldownThermalGate_018/LConn1
  HoldPipe_018/LConn2 -- HoldThermalGate_018/LConn1
  CooldownPipe_017/LConn2 -- CooldownThermalGate_017/LConn1
  HoldPipe_017/LConn2 -- HoldThermalGate_017/LConn1
  CooldownPipe_016/LConn2 -- CooldownThermalGate_016/LConn1
  HoldPipe_016/LConn2 -- HoldThermalGate_016/LConn1
  CooldownPipe_015/LConn2 -- CooldownThermalGate_015/LConn1
  HoldPipe_015/LConn2 -- HoldThermalGate_015/LConn1
  CooldownPipe_014/LConn2 -- CooldownThermalGate_014/LConn1
  HoldPipe_014/LConn2 -- HoldThermalGate_014/LConn1
  CooldownPipe_013/LConn2 -- CooldownThermalGate_013/LConn1
  HoldPipe_013/LConn2 -- HoldThermalGate_013/LConn1
  CooldownPipe_012/LConn2 -- CooldownThermalGate_012/LConn1
  HoldPipe_012/LConn2 -- HoldThermalGate_012/LConn1
  CooldownPipe_011/LConn2 -- CooldownThermalGate_011/LConn1
  HoldPipe_011/LConn2 -- HoldThermalGate_011/LConn1
  CooldownPipe_010/LConn2 -- CooldownThermalGate_010/LConn1
  HoldPipe_010/LConn2 -- HoldThermalGate_010/LConn1
  CooldownPipe_009/LConn2 -- CooldownThermalGate_009/LConn1
  HoldPipe_009/LConn2 -- HoldThermalGate_009/LConn1
  CooldownPipe_008/LConn2 -- CooldownThermalGate_008/LConn1
  HoldPipe_008/LConn2 -- HoldThermalGate_008/LConn1
  CooldownPipe_007/LConn2 -- CooldownThermalGate_007/LConn1
  HoldPipe_007/LConn2 -- HoldThermalGate_007/LConn1
  CooldownPipe_006/LConn2 -- CooldownThermalGate_006/LConn1
  HoldPipe_006/LConn2 -- HoldThermalGate_006/LConn1
  CooldownPipe_005/LConn2 -- CooldownThermalGate_005/LConn1
  HoldPipe_005/LConn2 -- HoldThermalGate_005/LConn1
  CooldownPipe_004/LConn2 -- CooldownThermalGate_004/LConn1
  HoldPipe_004/LConn2 -- HoldThermalGate_004/LConn1
  CooldownPipe_003/LConn2 -- CooldownThermalGate_003/LConn1
  HoldPipe_003/LConn2 -- HoldThermalGate_003/LConn1
  CooldownPipe_002/LConn2 -- CooldownThermalGate_002/LConn1
  HoldPipe_002/LConn2 -- HoldThermalGate_002/LConn1
  CooldownPipe_001/LConn2 -- CooldownThermalGate_001/LConn1
  HoldPipe_001/LConn2 -- HoldThermalGate_001/LConn1
  HoldThermalGateCommandPS/RConn1 -- HoldThermalGate_001/LConn2 -- HoldThermalGate_002/LConn2 -- HoldThermalGate_003/LConn2 -- HoldThermalGate_004/LConn2 -- HoldThermalGate_005/LConn2 -- HoldThermalGate_006/LConn2 -- HoldThermalGate_007/LConn2 -- HoldThermalGate_008/LConn2 -- HoldThermalGate_009/LConn2 -- HoldThermalGate_010/LConn2 -- HoldThermalGate_011/LConn2 -- HoldThermalGate_012/LConn2 -- HoldThermalGate_013/LConn2 -- HoldThermalGate_014/LConn2 -- HoldThermalGate_015/LConn2 -- HoldThermalGate_016/LConn2 -- HoldThermalGate_017/LConn2 -- HoldThermalGate_018/LConn2 -- HoldThermalGate_019/LConn2 -- HoldThermalGate_020/LConn2 -- HoldThermalGate_021/LConn2
  CooldownThermalGateCommandPS/RConn1 -- CooldownThermalGate_001/LConn2 -- CooldownThermalGate_002/LConn2 -- CooldownThermalGate_003/LConn2 -- CooldownThermalGate_004/LConn2 -- CooldownThermalGate_005/LConn2 -- CooldownThermalGate_006/LConn2 -- CooldownThermalGate_007/LConn2 -- CooldownThermalGate_008/LConn2 -- CooldownThermalGate_009/LConn2 -- CooldownThermalGate_010/LConn2 -- CooldownThermalGate_011/LConn2 -- CooldownThermalGate_012/LConn2 -- CooldownThermalGate_013/LConn2 -- CooldownThermalGate_014/LConn2 -- CooldownThermalGate_015/LConn2 -- CooldownThermalGate_016/LConn2 -- CooldownThermalGate_017/LConn2 -- CooldownThermalGate_018/LConn2 -- CooldownThermalGate_019/LConn2 -- CooldownThermalGate_020/LConn2 -- CooldownThermalGate_021/LConn2
  Conn2/RConn1 -- HoldPipe_001/LConn1 -- SMAHoldPipeNode01FluidTempSensor/LConn1
  SMAHoldPipeNode01FluidTempSensor/RConn2 -- SMAHoldPipeNode01FluidTempPS/LConn1
  SMAHoldPipeNode01FluidTempSensor/RConn1 -- SMAHoldPipeNode01FluidTempPressurePS/LConn1
  HoldPipe_010/RConn1 -- HoldPipe_011/LConn1 -- SMAHoldPipeNode11FluidTempSensor/LConn1
  SMAHoldPipeNode11FluidTempSensor/RConn2 -- SMAHoldPipeNode11FluidTempPS/LConn1
  SMAHoldPipeNode11FluidTempSensor/RConn1 -- SMAHoldPipeNode11FluidTempPressurePS/LConn1
  SMAHoldPipeNode21FluidTempSensor/RConn2 -- SMAHoldPipeNode21FluidTempPS/LConn1
  SMAHoldPipeNode21FluidTempSensor/RConn1 -- SMAHoldPipeNode21FluidTempPressurePS/LConn1
  CooldownPipe_001/RConn1 -- Conn3/RConn1 -- SMACooldownPipeNode01FluidTempSensor/LConn1
  SMACooldownPipeNode01FluidTempSensor/RConn2 -- SMACooldownPipeNode01FluidTempPS/LConn1
  SMACooldownPipeNode01FluidTempSensor/RConn1 -- SMACooldownPipeNode01FluidTempPressurePS/LConn1
  CooldownPipe_012/RConn1 -- CooldownPipe_011/LConn1 -- SMACooldownPipeNode11FluidTempSensor/LConn1
  SMACooldownPipeNode11FluidTempSensor/RConn2 -- SMACooldownPipeNode11FluidTempPS/LConn1
  SMACooldownPipeNode11FluidTempSensor/RConn1 -- SMACooldownPipeNode11FluidTempPressurePS/LConn1
  Conn4/RConn1 -- CooldownPipe_021/LConn1 -- SMACooldownPipeNode21FluidTempSensor/LConn1
  SMACooldownPipeNode21FluidTempSensor/RConn2 -- SMACooldownPipeNode21FluidTempPS/LConn1
  SMACooldownPipeNode21FluidTempSensor/RConn1 -- SMACooldownPipeNode21FluidTempPressurePS/LConn1
  HoldThermalGate_001/RConn1 -- SMAHoldNode01HeatFlowSensor/LConn1
  SMAHoldNode01HeatFlowSensor/RConn2 -- Subsystem2/RConn1
  SMAHoldNode01HeatFlowSensor/RConn1 -- SMAHoldNode01HeatFlowPS/LConn1
  HoldThermalGate_002/RConn1 -- SMAHoldNode02HeatFlowSensor/LConn1
  SMAHoldNode02HeatFlowSensor/RConn2 -- Subsystem2/RConn2
  SMAHoldNode02HeatFlowSensor/RConn1 -- SMAHoldNode02HeatFlowPS/LConn1
  HoldThermalGate_003/RConn1 -- SMAHoldNode03HeatFlowSensor/LConn1
  SMAHoldNode03HeatFlowSensor/RConn2 -- Subsystem2/RConn3
  SMAHoldNode03HeatFlowSensor/RConn1 -- SMAHoldNode03HeatFlowPS/LConn1
  HoldThermalGate_004/RConn1 -- SMAHoldNode04HeatFlowSensor/LConn1
  SMAHoldNode04HeatFlowSensor/RConn2 -- Subsystem2/RConn4
  SMAHoldNode04HeatFlowSensor/RConn1 -- SMAHoldNode04HeatFlowPS/LConn1
  HoldThermalGate_005/RConn1 -- SMAHoldNode05HeatFlowSensor/LConn1
  SMAHoldNode05HeatFlowSensor/RConn2 -- Subsystem2/RConn5
  SMAHoldNode05HeatFlowSensor/RConn1 -- SMAHoldNode05HeatFlowPS/LConn1
  HoldThermalGate_006/RConn1 -- SMAHoldNode06HeatFlowSensor/LConn1
  SMAHoldNode06HeatFlowSensor/RConn2 -- Subsystem2/RConn6
  SMAHoldNode06HeatFlowSensor/RConn1 -- SMAHoldNode06HeatFlowPS/LConn1
  HoldThermalGate_007/RConn1 -- SMAHoldNode07HeatFlowSensor/LConn1
  SMAHoldNode07HeatFlowSensor/RConn2 -- Subsystem2/RConn7
  SMAHoldNode07HeatFlowSensor/RConn1 -- SMAHoldNode07HeatFlowPS/LConn1
  HoldThermalGate_008/RConn1 -- SMAHoldNode08HeatFlowSensor/LConn1
  SMAHoldNode08HeatFlowSensor/RConn2 -- Subsystem2/RConn8
  SMAHoldNode08HeatFlowSensor/RConn1 -- SMAHoldNode08HeatFlowPS/LConn1
  HoldThermalGate_009/RConn1 -- SMAHoldNode09HeatFlowSensor/LConn1
  SMAHoldNode09HeatFlowSensor/RConn2 -- Subsystem2/RConn9
  SMAHoldNode09HeatFlowSensor/RConn1 -- SMAHoldNode09HeatFlowPS/LConn1
  HoldThermalGate_010/RConn1 -- SMAHoldNode10HeatFlowSensor/LConn1
  SMAHoldNode10HeatFlowSensor/RConn2 -- Subsystem2/RConn10
  SMAHoldNode10HeatFlowSensor/RConn1 -- SMAHoldNode10HeatFlowPS/LConn1
  HoldThermalGate_011/RConn1 -- SMAHoldNode11HeatFlowSensor/LConn1
  SMAHoldNode11HeatFlowSensor/RConn2 -- Subsystem2/RConn11
  SMAHoldNode11HeatFlowSensor/RConn1 -- SMAHoldNode11HeatFlowPS/LConn1
  HoldThermalGate_012/RConn1 -- SMAHoldNode12HeatFlowSensor/LConn1
  SMAHoldNode12HeatFlowSensor/RConn2 -- Subsystem2/RConn12
  SMAHoldNode12HeatFlowSensor/RConn1 -- SMAHoldNode12HeatFlowPS/LConn1
  HoldThermalGate_013/RConn1 -- SMAHoldNode13HeatFlowSensor/LConn1
  SMAHoldNode13HeatFlowSensor/RConn2 -- Subsystem2/RConn13
  SMAHoldNode13HeatFlowSensor/RConn1 -- SMAHoldNode13HeatFlowPS/LConn1
  HoldThermalGate_014/RConn1 -- SMAHoldNode14HeatFlowSensor/LConn1
  SMAHoldNode14HeatFlowSensor/RConn2 -- Subsystem2/RConn14
  SMAHoldNode14HeatFlowSensor/RConn1 -- SMAHoldNode14HeatFlowPS/LConn1
  HoldThermalGate_015/RConn1 -- SMAHoldNode15HeatFlowSensor/LConn1
  SMAHoldNode15HeatFlowSensor/RConn2 -- Subsystem2/RConn15
  SMAHoldNode15HeatFlowSensor/RConn1 -- SMAHoldNode15HeatFlowPS/LConn1
  HoldThermalGate_016/RConn1 -- SMAHoldNode16HeatFlowSensor/LConn1
  SMAHoldNode16HeatFlowSensor/RConn2 -- Subsystem2/RConn16
  SMAHoldNode16HeatFlowSensor/RConn1 -- SMAHoldNode16HeatFlowPS/LConn1
  HoldThermalGate_017/RConn1 -- SMAHoldNode17HeatFlowSensor/LConn1
  SMAHoldNode17HeatFlowSensor/RConn2 -- Subsystem2/RConn17
  SMAHoldNode17HeatFlowSensor/RConn1 -- SMAHoldNode17HeatFlowPS/LConn1
  HoldThermalGate_018/RConn1 -- SMAHoldNode18HeatFlowSensor/LConn1
  SMAHoldNode18HeatFlowSensor/RConn2 -- Subsystem2/RConn18
  SMAHoldNode18HeatFlowSensor/RConn1 -- SMAHoldNode18HeatFlowPS/LConn1
  HoldThermalGate_019/RConn1 -- SMAHoldNode19HeatFlowSensor/LConn1
  SMAHoldNode19HeatFlowSensor/RConn2 -- Subsystem2/RConn19
  SMAHoldNode19HeatFlowSensor/RConn1 -- SMAHoldNode19HeatFlowPS/LConn1
  HoldThermalGate_020/RConn1 -- SMAHoldNode20HeatFlowSensor/LConn1
  SMAHoldNode20HeatFlowSensor/RConn2 -- Subsystem2/RConn20
  SMAHoldNode20HeatFlowSensor/RConn1 -- SMAHoldNode20HeatFlowPS/LConn1
  HoldThermalGate_021/RConn1 -- SMAHoldNode21HeatFlowSensor/LConn1
  SMAHoldNode21HeatFlowSensor/RConn2 -- Subsystem2/RConn21
  SMAHoldNode21HeatFlowSensor/RConn1 -- SMAHoldNode21HeatFlowPS/LConn1
  CooldownThermalGate_001/RConn1 -- SMACooldownNode01HeatFlowSensor/LConn1
  SMACooldownNode01HeatFlowSensor/RConn2 -- Subsystem2/RConn22
  SMACooldownNode01HeatFlowSensor/RConn1 -- SMACooldownNode01HeatFlowPS/LConn1
  CooldownThermalGate_002/RConn1 -- SMACooldownNode02HeatFlowSensor/LConn1
  SMACooldownNode02HeatFlowSensor/RConn2 -- Subsystem2/RConn23
  SMACooldownNode02HeatFlowSensor/RConn1 -- SMACooldownNode02HeatFlowPS/LConn1
  CooldownThermalGate_003/RConn1 -- SMACooldownNode03HeatFlowSensor/LConn1
  SMACooldownNode03HeatFlowSensor/RConn2 -- Subsystem2/RConn24
  SMACooldownNode03HeatFlowSensor/RConn1 -- SMACooldownNode03HeatFlowPS/LConn1
  CooldownThermalGate_004/RConn1 -- SMACooldownNode04HeatFlowSensor/LConn1
  SMACooldownNode04HeatFlowSensor/RConn2 -- Subsystem2/RConn25
  SMACooldownNode04HeatFlowSensor/RConn1 -- SMACooldownNode04HeatFlowPS/LConn1
  CooldownThermalGate_005/RConn1 -- SMACooldownNode05HeatFlowSensor/LConn1
  SMACooldownNode05HeatFlowSensor/RConn2 -- Subsystem2/RConn26
  SMACooldownNode05HeatFlowSensor/RConn1 -- SMACooldownNode05HeatFlowPS/LConn1
  CooldownThermalGate_006/RConn1 -- SMACooldownNode06HeatFlowSensor/LConn1
  SMACooldownNode06HeatFlowSensor/RConn2 -- Subsystem2/RConn27
  SMACooldownNode06HeatFlowSensor/RConn1 -- SMACooldownNode06HeatFlowPS/LConn1
  CooldownThermalGate_007/RConn1 -- SMACooldownNode07HeatFlowSensor/LConn1
  SMACooldownNode07HeatFlowSensor/RConn2 -- Subsystem2/RConn28
  SMACooldownNode07HeatFlowSensor/RConn1 -- SMACooldownNode07HeatFlowPS/LConn1
  CooldownThermalGate_008/RConn1 -- SMACooldownNode08HeatFlowSensor/LConn1
  SMACooldownNode08HeatFlowSensor/RConn2 -- Subsystem2/RConn29
  SMACooldownNode08HeatFlowSensor/RConn1 -- SMACooldownNode08HeatFlowPS/LConn1
  CooldownThermalGate_009/RConn1 -- SMACooldownNode09HeatFlowSensor/LConn1
  SMACooldownNode09HeatFlowSensor/RConn2 -- Subsystem2/RConn30
  SMACooldownNode09HeatFlowSensor/RConn1 -- SMACooldownNode09HeatFlowPS/LConn1
  CooldownThermalGate_010/RConn1 -- SMACooldownNode10HeatFlowSensor/LConn1
  SMACooldownNode10HeatFlowSensor/RConn2 -- Subsystem2/RConn31
  SMACooldownNode10HeatFlowSensor/RConn1 -- SMACooldownNode10HeatFlowPS/LConn1
  CooldownThermalGate_011/RConn1 -- SMACooldownNode11HeatFlowSensor/LConn1
  SMACooldownNode11HeatFlowSensor/RConn2 -- Subsystem2/RConn32
  SMACooldownNode11HeatFlowSensor/RConn1 -- SMACooldownNode11HeatFlowPS/LConn1
  CooldownThermalGate_012/RConn1 -- SMACooldownNode12HeatFlowSensor/LConn1
  SMACooldownNode12HeatFlowSensor/RConn2 -- Subsystem2/RConn33
  SMACooldownNode12HeatFlowSensor/RConn1 -- SMACooldownNode12HeatFlowPS/LConn1
  CooldownThermalGate_013/RConn1 -- SMACooldownNode13HeatFlowSensor/LConn1
  SMACooldownNode13HeatFlowSensor/RConn2 -- Subsystem2/RConn34
  SMACooldownNode13HeatFlowSensor/RConn1 -- SMACooldownNode13HeatFlowPS/LConn1
  CooldownThermalGate_014/RConn1 -- SMACooldownNode14HeatFlowSensor/LConn1
  SMACooldownNode14HeatFlowSensor/RConn2 -- Subsystem2/RConn35
  SMACooldownNode14HeatFlowSensor/RConn1 -- SMACooldownNode14HeatFlowPS/LConn1
  CooldownThermalGate_015/RConn1 -- SMACooldownNode15HeatFlowSensor/LConn1
  SMACooldownNode15HeatFlowSensor/RConn2 -- Subsystem2/RConn36
  SMACooldownNode15HeatFlowSensor/RConn1 -- SMACooldownNode15HeatFlowPS/LConn1
  CooldownThermalGate_016/RConn1 -- SMACooldownNode16HeatFlowSensor/LConn1
  SMACooldownNode16HeatFlowSensor/RConn2 -- Subsystem2/RConn37
  SMACooldownNode16HeatFlowSensor/RConn1 -- SMACooldownNode16HeatFlowPS/LConn1
  CooldownThermalGate_017/RConn1 -- SMACooldownNode17HeatFlowSensor/LConn1
  SMACooldownNode17HeatFlowSensor/RConn2 -- Subsystem2/RConn38
  SMACooldownNode17HeatFlowSensor/RConn1 -- SMACooldownNode17HeatFlowPS/LConn1
  CooldownThermalGate_018/RConn1 -- SMACooldownNode18HeatFlowSensor/LConn1
  SMACooldownNode18HeatFlowSensor/RConn2 -- Subsystem2/RConn39
  SMACooldownNode18HeatFlowSensor/RConn1 -- SMACooldownNode18HeatFlowPS/LConn1
  CooldownThermalGate_019/RConn1 -- SMACooldownNode19HeatFlowSensor/LConn1
  SMACooldownNode19HeatFlowSensor/RConn2 -- Subsystem2/RConn40
  SMACooldownNode19HeatFlowSensor/RConn1 -- SMACooldownNode19HeatFlowPS/LConn1
  CooldownThermalGate_020/RConn1 -- SMACooldownNode20HeatFlowSensor/LConn1
  SMACooldownNode20HeatFlowSensor/RConn2 -- Subsystem2/RConn41
  SMACooldownNode20HeatFlowSensor/RConn1 -- SMACooldownNode20HeatFlowPS/LConn1
  CooldownThermalGate_021/RConn1 -- SMACooldownNode21HeatFlowSensor/LConn1
  SMACooldownNode21HeatFlowSensor/RConn2 -- Subsystem2/RConn42
  SMACooldownNode21HeatFlowSensor/RConn1 -- SMACooldownNode21HeatFlowPS/LConn1
